simulink model "FullFMS_SIM_V0_1_8_R2025b"  (R2025b)
settings: Solver=FixedStepAuto  StopTime=inf  FixedStep=0.01  MaxStep=0.01  RelTol=1e-2
PreLoadFcn:
  | load("BUS_CONFIG_SIM.mat"); run("Param_SIM_V0_1_8.m")
libraries: opcualib x8
(part 2 of 2)

== stateflow chart FullFMS_SIM_V0_1_8_R2025b/Chart_SIM ==
  settings: updateMethod=DISCRETE  sampleTime=Ts_SIM
  state HD1_Ctrl [parallel]
    settings: executionOrder=2
    state Init
      entry: SimControl_50.SC_52_Profibus=true; SimControl_50.SC_55_PD_Sort=false; SimASi_50.SR_54_CRoute_Out=false;
      SimActuators_50.SA_50_Claw_Down=false; SimActuators_50.SA_50_Close_Claw=false; SimActuators_50.SA_50_Claw_2_Del=false; SimActuators_50.SA_50_Claw_2_Cart=false;
    state Ready
      entry: SimControl_50.SC_55_Initialization=true;
    state N1_StartMove
      entry: SimControl_50.SC_55_PD_Sort=false;
    state N2_LowerClaw
      entry: SimActuators_50.SA_50_Claw_Down=true;
    state N3_CloseClaw
      entry: SimActuators_50.SA_50_Close_Claw=true;
    state N3_Raise
      entry: SimActuators_50.SA_50_Claw_Down=false;
    state N4_Claw2Del
      entry: SimActuators_50.SA_50_Claw_2_Cart=false; SimActuators_50.SA_50_Claw_2_Del=true;
    state N5_LowerClaw2
      entry: SimActuators_50.SA_50_Claw_Down=true;
    state N6_Release
      entry: SimActuators_50.SA_50_Close_Claw=false;
    state N6_Raise
      entry: SimActuators_50.SA_50_Claw_Down=false;
    state N7_PDSort
      entry: SimControl_50.SC_55_PD_Sort=true;
    state N8_Claw2Cart
      entry: SimActuators_50.SA_50_Claw_2_Del=false; SimActuators_50.SA_50_Claw_2_Cart=true; Claw2CartCmd=true;
    state N9_CRouteOut
      entry: SimActuators_50.SA_50_Claw_2_Cart=false; Claw2CartCmd=false; RouteOut54=true; SimASi_50.SR_54_CRoute_Out=true;
      exit: RouteOut54=false; SimASi_50.SR_54_CRoute_Out=false; nCart = nCart + 1;
    (default) -> Init
    Init -> Ready : [SimSensors_50.SS_50_Claw_Cart && SimSensors_50.SS_50_Claw_High && ~SimSensors_50.SS_50_Part_in_Claw]
    N9_CRouteOut -> Ready : after(T_HD1_T1,sec)
    Ready -> N1_StartMove : [CRouteIn54 && CartAt29 && SimSensors_20.SS_29_Optic && ~SimSensors_60.SS_60_SPart]
    N1_StartMove -> N2_LowerClaw : [~SimControl_50.SC_55_PD_Sort && SimSensors_50.SS_50_Claw_Cart && SimSensors_50.SS_50_Claw_High && ~SimSensors_50.SS_50_Part_in_Claw]
    N2_LowerClaw -> N3_CloseClaw : [SimSensors_50.SS_50_Claw_Cart && SimSensors_50.SS_50_Claw_Low]
    N3_CloseClaw -> N3_Raise : [SimSensors_50.SS_50_Part_in_Claw]
    N3_Raise -> N4_Claw2Del : [SimSensors_50.SS_50_Claw_High && SimSensors_50.SS_50_Part_in_Claw && ~SimSensors_50.SS_50_Claw_Del]
    N4_Claw2Del -> N5_LowerClaw2 : [SimSensors_50.SS_50_Claw_Del && SimSensors_50.SS_50_Claw_High && SimSensors_50.SS_50_Part_in_Claw]
    N5_LowerClaw2 -> N6_Release : [SimSensors_50.SS_50_Claw_Del && SimSensors_50.SS_50_Claw_Low]
    N6_Release -> N6_Raise : [~SimSensors_50.SS_50_Part_in_Claw]
    N6_Raise -> N7_PDSort : [SimSensors_50.SS_50_Claw_Del && SimSensors_50.SS_50_Claw_High && ~SimSensors_50.SS_50_Part_in_Claw]
    N7_PDSort -> N8_Claw2Cart
    N8_Claw2Cart -> N9_CRouteOut : [SimSensors_50.SS_50_Claw_Cart]
  state HD1_Plant [parallel]
    settings: executionOrder=3
    state Vertical [parallel]
      settings: executionOrder=1
      state High
        entry: SimSensors_50.SS_50_Claw_High=true; SimSensors_50.SS_50_Claw_Low=false;
      state GoingDown
        entry: SimSensors_50.SS_50_Claw_High=false;
      state Low
        entry: SimSensors_50.SS_50_Claw_Low=true;
      state GoingUp
        entry: SimSensors_50.SS_50_Claw_Low=false;
      (default) -> High
      GoingUp -> High [order 1] : after(t_v_up,sec)
      High -> GoingDown : [SimActuators_50.SA_50_Claw_Down]
      GoingUp -> GoingDown [order 2] : [SimActuators_50.SA_50_Claw_Down]
      GoingDown -> Low [order 1] : after(t_v_down,sec)
      GoingDown -> GoingUp [order 2] : [~SimActuators_50.SA_50_Claw_Down]
      Low -> GoingUp : [~SimActuators_50.SA_50_Claw_Down]
    state Horizontal [parallel]
      settings: executionOrder=2
      state AtCart
        entry: SimSensors_50.SS_50_Claw_Cart=true; SimSensors_50.SS_50_Claw_Del=false;
      state ToDel
        entry: SimSensors_50.SS_50_Claw_Cart=false;
      state AtDel
        entry: SimSensors_50.SS_50_Claw_Del=true;
      state ToCart
        entry: SimSensors_50.SS_50_Claw_Del=false;
      (default) -> AtCart
      ToCart -> AtCart : after(t_h_cart,sec)
      AtCart -> ToDel : [SimActuators_50.SA_50_Claw_2_Del]
      ToDel -> AtDel : after(t_h_del,sec)
      AtDel -> ToCart : [SimActuators_50.SA_50_Claw_2_Cart]
    state Gripper [parallel]
      settings: executionOrder=3
      state Empty
        entry: SimSensors_50.SS_50_Part_in_Claw=false;
      state Gripping
      state Holding
        entry: SimSensors_50.SS_50_Part_in_Claw=true; cartPart=false;
      state Releasing
      (default) -> HD1_Plant.Gripper.Empty
      Releasing -> HD1_Plant.Gripper.Empty : after(t_grip,sec){SimSensors_60.SS_60_SPart = SimSensors_60.SS_60_SPart || SimSensors_50.SS_50_Claw_Del;}
      HD1_Plant.Gripper.Empty -> Gripping : [SimActuators_50.SA_50_Close_Claw && SimSensors_50.SS_50_Claw_Low && SimSensors_50.SS_50_Claw_Cart && PartOnCart]
      Gripping -> Holding : after(t_grip,sec)
      Holding -> Releasing : [~SimActuators_50.SA_50_Close_Claw && SimSensors_50.SS_50_Claw_Low]
  state SORT_Ctrl [parallel]
    entry: SimControl_60.SC_62_Profibus=false; SimControl_60.SC_65_Initialization=false; SimControl_60.SC_65_ID_1=false; SimControl_60.SC_65_ID_2=false; SimControl_60.SC_65_Part_Sorted=false;
    SimControl_60.SC_65_RBS_Output = (SORT_MODE == 1); SimControl_60.SC_65_RSB_Output = (SORT_MODE == 2); SimControl_60.SC_65_BRS_Output = (SORT_MODE == 3); SimControl_60.SC_65_BSR_Output = (SORT_MODE == 4); SimControl_60.SC_65_SRB_Output = (SORT_MODE == 5); SimControl_60.SC_65_SBR_Output = (SORT_MODE == 6);
    SimActuators_60.SA_60_Conveyor=false; SimActuators_60.SA_60_P1=false; SimActuators_60.SA_60_P2=false; SimActuators_60.SA_60_Identify=false; SimActuators_60.SA_61_Led_Start=false; SimActuators_60.SA_61_Led_Reset=false; SimActuators_60.SA_61_Led_Extra1=false; SimActuators_60.SA_61_Led_Extra2=false; SimActuators_60.SA_61_Panel_O4=false; SimActuators_60.SA_61_Panel_O5=false; SimActuators_60.SA_61_Panel_O6=false; SimActuators_60.SA_61_Panel_O7=false;
    FBSel = (SORT_MODE == 1 && SimControl_60.SC_65_RBS_Output) || (SORT_MODE == 2 && SimControl_60.SC_65_RSB_Output) || (SORT_MODE == 3 && SimControl_60.SC_65_BRS_Output) || (SORT_MODE == 4 && SimControl_60.SC_65_BSR_Output) || (SORT_MODE == 5 && SimControl_60.SC_65_SRB_Output) || (SORT_MODE == 6 && SimControl_60.SC_65_SBR_Output);
    settings: executionOrder=5
    state FB1_Init [parallel]
      settings: executionOrder=1
      state FB1_N2_Check
        entry: SimControl_60.SC_62_Profibus=true; FB1Init=false; SimControl_60.SC_65_Initialization=false;
      state FB1_N3_ClearPart
        entry: FB1Conv=true; FB1IDPin=true;
      state FB1_N1_InitOk
        entry: FB1Init=true; SimControl_60.SC_65_Initialization=true;
      (default) -> SORT_Ctrl.FB1_Init.FB1_N2_Check
      FB1_N3_ClearPart -> SORT_Ctrl.FB1_Init.FB1_N2_Check : [FB1Conv && SimSensors_60.SS_60_Part_Pass]{FB1Conv=false; FB1IDPin=false;}
      SORT_Ctrl.FB1_Init.FB1_N1_InitOk -> SORT_Ctrl.FB1_Init.FB1_N2_Check : [SimSensors_60.SS_61_Reset]{FB1Conv=false; FB1IDPin=false; TrigConv=false; Lever1=false; Lever2=false; PinSort=false; PartDel=false;}
      SORT_Ctrl.FB1_Init.FB1_N2_Check -> SORT_Ctrl.FB1_Init.FB1_N1_InitOk [order 1] : [SimControl_60.SC_62_Profibus && ~FB1Conv && ~SimSensors_60.SS_60_SPart && ~SimSensors_60.SS_60_SInd && ~SimSensors_60.SS_60_SPhoto && ~SimSensors_60.SS_60_Part_Pass]
      SORT_Ctrl.FB1_Init.FB1_N2_Check -> FB1_N3_ClearPart [order 2] : [SimSensors_60.SS_60_SPart || SimSensors_60.SS_60_SInd || SimSensors_60.SS_60_SPhoto]
    state FB4_9_Sort [parallel]
      settings: executionOrder=2
      state OB1_N4_9_Select
      state N1_StartConv
        entry: TrigConv=true; SimControl_60.SC_65_ID_1=false; SimControl_60.SC_65_ID_2=false;
      state N2_Identify
        en, du: if SimSensors_60.SS_60_SInd, SimControl_60.SC_65_ID_1=false; SimControl_60.SC_65_ID_2=true;
        elseif SimSensors_60.SS_60_SPhoto, SimControl_60.SC_65_ID_1=true; SimControl_60.SC_65_ID_2=true;
        else, SimControl_60.SC_65_ID_1=true; SimControl_60.SC_65_ID_2=false; end
      state N3_SelectLever
        entry: cID = 0;
        if SimControl_60.SC_65_ID_1 && SimControl_60.SC_65_ID_2, cID = 1; elseif SimControl_60.SC_65_ID_1, cID = 2; elseif SimControl_60.SC_65_ID_2, cID = 3; end
        Lever1 = (cID == SORT_MAP(SORT_MODE,1)); Lever2 = (cID == SORT_MAP(SORT_MODE,2)); PassStr = (cID == SORT_MAP(SORT_MODE,3));
        during: if (Lever1 && SimSensors_60.SS_60_SL1_Fwd) || (Lever2 && SimSensors_60.SS_60_SL2_Fwd) || (PassStr && SimSensors_60.SS_60_SL1_Bck && SimSensors_60.SS_60_SL2_Bck), PinSort = true; end
      state N4_PartDel
        entry: PartDel=true; Lever1=false;
        if SORT_MODE ~= 3, Lever2=false; end
      state N5_ResetNext
        entry: TrigConv=false; PinSort=false; PartDel=false; Lever1=false; Lever2=false; PassStr=false;
      (default) -> OB1_N4_9_Select
      N5_ResetNext -> OB1_N4_9_Select
      OB1_N4_9_Select -> N1_StartConv : [FB1Init && FBSel && SimControl_50.SC_55_PD_Sort && SimSensors_50.SS_50_Claw_Del]
      N1_StartConv -> N2_Identify
      N2_Identify -> N3_SelectLever : after(T_SORT_ID - Ts_SIM,sec)
      N3_SelectLever -> N4_PartDel : [SimSensors_60.SS_60_Part_Pass]
      N4_PartDel -> N5_ResetNext
    state OB1_N10_11 [parallel]
      settings: executionOrder=3
      state N10_Wait
        entry: SimControl_60.SC_65_Part_Sorted=false;
      state N10_PartPass
      state N11_PartSorted
        entry: SimControl_60.SC_65_Part_Sorted=true;
      (default) -> N10_Wait
      N11_PartSorted -> N10_Wait : after(T_SORT_T7,sec)
      N10_Wait -> N10_PartPass : [SimSensors_60.SS_60_Part_Pass]
      N10_PartPass -> N11_PartSorted : [~SimSensors_60.SS_60_Part_Pass]
    state FB3_Actuators [parallel]
      settings: executionOrder=4
      state FB3_Map
        during: ConvOn60 = SimSensors_60.SS_61_Key_Pos && (TrigConv || FB1Conv); SimActuators_60.SA_60_Conveyor = ConvOn60;
        SimActuators_60.SA_60_P1 = SimSensors_60.SS_61_Key_Pos && Lever1; SimActuators_60.SA_60_P2 = SimSensors_60.SS_61_Key_Pos && Lever2;
        SimActuators_60.SA_60_Identify = SimSensors_60.SS_61_Key_Pos && (PinSort || FB1IDPin);
        SimActuators_60.SA_61_Led_Start = SimSensors_60.SS_61_Key_Pos && FB1Init; SimActuators_60.SA_61_Led_Reset = SimSensors_60.SS_61_Key_Pos && SimSensors_60.SS_61_Reset;
        SimActuators_60.SA_61_Led_Extra1 = SimControl_60.SC_65_Part_Sorted; SimActuators_60.SA_61_Led_Extra2 = false;
        SimActuators_60.SA_61_Panel_O4 = false; SimActuators_60.SA_61_Panel_O5 = false; SimActuators_60.SA_61_Panel_O6 = false; SimActuators_60.SA_61_Panel_O7 = false;
      (default) -> SORT_Ctrl.FB3_Actuators.FB3_Map
  state SORT_Plant [parallel]
    entry: SimSensors_60.SS_60_SPart=false; SimSensors_60.SS_60_SInd=false; SimSensors_60.SS_60_SPhoto=false; SimSensors_60.SS_60_Part_Pass=false;
    SimSensors_60.SS_60_SL1_Bck=true; SimSensors_60.SS_60_SL1_Fwd=false; SimSensors_60.SS_60_SL2_Bck=true; SimSensors_60.SS_60_SL2_Fwd=false;
    SimSensors_60.SS_61_Key_Pos=true; SimSensors_60.SS_61_Start=false; SimSensors_60.SS_61_Stop=false; SimSensors_60.SS_61_Reset=false;
    SimSensors_60.SS_61_Panel_I4=false; SimSensors_60.SS_61_Panel_I5=false; SimSensors_60.SS_61_Panel_I6=false; SimSensors_60.SS_61_Panel_I7=false;
    settings: executionOrder=4
    state Part [parallel]
      settings: executionOrder=1
      state Empty
        entry: SimSensors_60.SS_60_Part_Pass=false;
      state AtEntry
        entry: sortColor = PART_COLORS(min(nSortIn+1, numel(PART_COLORS))); nSortIn = nSortIn + 1;
      state ToStopper
        entry: xSort = 0;
        during: if ConvOn60, xSort = xSort + Ts_SIM; end
        SimSensors_60.SS_60_SPart = xSort < t_s_spart_off;
        if xSort >= t_s_photo, SimSensors_60.SS_60_SPhoto = (sortColor ~= 2); end
        if xSort >= t_s_ind, SimSensors_60.SS_60_SInd = (sortColor == 3); end
      state AtStopper
      state Released
        entry: xSort = 0;
        if SimSensors_60.SS_60_SL1_Fwd, sortExit = 1; elseif SimSensors_60.SS_60_SL2_Fwd, sortExit = 2; else, sortExit = 3; end
        during: if ConvOn60, xSort = xSort + Ts_SIM; end
        if xSort >= t_s_ind_off, SimSensors_60.SS_60_SInd = false; end
        if xSort >= t_s_photo_off, SimSensors_60.SS_60_SPhoto = false; end
      state PartPass
        entry: SimSensors_60.SS_60_Part_Pass = true; SimSensors_60.SS_60_SInd = false; SimSensors_60.SS_60_SPhoto = false; nDone = nDone + 1;
      (default) -> SORT_Plant.Part.Empty
      PartPass -> SORT_Plant.Part.Empty : after(t_s_pp,sec)
      SORT_Plant.Part.Empty -> AtEntry : [SimSensors_60.SS_60_SPart]
      AtEntry -> ToStopper : [SimActuators_60.SA_60_Conveyor]
      ToStopper -> AtStopper : [xSort >= t_s_ind]
      AtStopper -> Released : [SimActuators_60.SA_60_Identify && SimActuators_60.SA_60_Conveyor]
      Released -> PartPass : [(sortExit == 1 && xSort >= t_s_pass1) || (sortExit == 2 && xSort >= t_s_pass2) || (sortExit == 3 && xSort >= t_s_pass3)]
    state Lever1 [parallel]
      settings: executionOrder=2
      state SL1_Bck
        entry: SimSensors_60.SS_60_SL1_Bck=true; SimSensors_60.SS_60_SL1_Fwd=false;
      state SL1_ToFwd
        entry: SimSensors_60.SS_60_SL1_Bck=false;
      state SL1_Fwd
        entry: SimSensors_60.SS_60_SL1_Fwd=true;
      state SL1_ToBck
        entry: SimSensors_60.SS_60_SL1_Fwd=false;
      (default) -> SL1_Bck
      SL1_ToBck -> SL1_Bck [order 1] : after(t_sl1_bck,sec)
      SL1_Bck -> SL1_ToFwd : [SimActuators_60.SA_60_P1]
      SL1_ToBck -> SL1_ToFwd [order 2] : [SimActuators_60.SA_60_P1]
      SL1_ToFwd -> SL1_Fwd [order 1] : after(t_sl1_fwd,sec)
      SL1_ToFwd -> SL1_ToBck [order 2] : [~SimActuators_60.SA_60_P1]
      SL1_Fwd -> SL1_ToBck : [~SimActuators_60.SA_60_P1]
    state Lever2 [parallel]
      settings: executionOrder=3
      state SL2_Bck
        entry: SimSensors_60.SS_60_SL2_Bck=true; SimSensors_60.SS_60_SL2_Fwd=false;
      state SL2_ToFwd
        entry: SimSensors_60.SS_60_SL2_Bck=false;
      state SL2_Fwd
        entry: SimSensors_60.SS_60_SL2_Fwd=true;
      state SL2_ToBck
        entry: SimSensors_60.SS_60_SL2_Fwd=false;
      (default) -> SL2_Bck
      SL2_ToBck -> SL2_Bck [order 1] : after(t_sl2_bck,sec)
      SL2_Bck -> SL2_ToFwd : [SimActuators_60.SA_60_P2]
      SL2_ToBck -> SL2_ToFwd [order 2] : [SimActuators_60.SA_60_P2]
      SL2_ToFwd -> SL2_Fwd [order 1] : after(t_sl2_fwd,sec)
      SL2_ToFwd -> SL2_ToBck [order 2] : [~SimActuators_60.SA_60_P2]
      SL2_Fwd -> SL2_ToBck : [~SimActuators_60.SA_60_P2]
  state TEST_Ctrl [parallel]
    entry: SimControl_70.SC_72_Profibus=false; SimControl_70.SC_75_Initialization=false; SimControl_70.SC_75_RQ_Delivery1=false; SimControl_70.SC_75_ID_Delivery1=false; SimControl_70.SC_75_RQ_Delivery2=false; SimControl_70.SC_75_ID_Delivery2=false; SimControl_70.SC_75_Part_Del=false; SimControl_70.SC_75_RQ_Part_Del=false; SimControl_70.SC_75_RQ_Wrong=false;
    SimControl_70.SC_75_Identified = (TEST_MODE == 1); SimControl_70.SC_75_Requested = (TEST_MODE == 2); SimControl_70.SC_75_Identified80 = (TEST_MODE == 1); SimControl_70.SC_75_Requested80 = (TEST_MODE == 2);
    SimActuators_70.SA_70_Elev_Down=false; SimActuators_70.SA_70_Elev_Up=false; SimActuators_70.SA_70_Eject_Part=false; SimActuators_70.SA_70_Air_On=false; SimActuators_70.SA_71_Led_Start=false; SimActuators_70.SA_71_Led_Reset=false; SimActuators_70.SA_71_Led_Extra1=false; SimActuators_70.SA_71_Led_Extra2=false; SimActuators_70.SA_71_Panel_O4=false; SimActuators_70.SA_71_Panel_O5=false; SimActuators_70.SA_71_Panel_O6=false; SimActuators_70.SA_71_Panel_O7=false;
    SimASi_70.SR_73_TestCartID=0; SimASi_70.SR_74_Request=false; SimASi_70.SR_74_No_Cart=true; SimASi_70.SR_74_Cart_Full=false; SimASi_70.SR_74_CRoute_Out=false; SimASi_70.SR_74_CRoute_In=false;
    settings: executionOrder=6
    state FB1_Init70 [parallel]
      settings: executionOrder=1
      state FB1_N2_N3_Check
        entry: SimControl_70.SC_72_Profibus=true; FB1Init70=false; SimControl_70.SC_75_Initialization=false;
        during: FB1ElevDown70 = ~ElevLow70;
      state FB1_N3_PistonPulse
        entry: FB1PistAdv70=true;
      state FB1_N1_N4_InitOk
        entry: FB1Init70=true; SimControl_70.SC_75_Initialization=true; FB1ElevDown70=false; FB1PistAdv70=false;
      (default) -> TEST_Ctrl.FB1_Init70.FB1_N2_N3_Check
      FB1_N3_PistonPulse -> TEST_Ctrl.FB1_Init70.FB1_N2_N3_Check : after(T_TEST_T1,sec){FB1PistAdv70=false;}
      FB1_N1_N4_InitOk -> TEST_Ctrl.FB1_Init70.FB1_N2_N3_Check : [SimSensors_70.SS_71_Reset]{IdenDel=false; IdenProc=false; EjectProc=false; ReturnElev=false; ReqDel=false; IdenColor=false; PartOk=false; EjectOk=false; PartDiff=false; EjectBad=false;}
      TEST_Ctrl.FB1_Init70.FB1_N2_N3_Check -> FB1_N1_N4_InitOk [order 1] : [~PartIn70 && ElevLow70 && PistBck70 && DistInit85]
      TEST_Ctrl.FB1_Init70.FB1_N2_N3_Check -> FB1_N3_PistonPulse [order 2] : [ElevLow70 && PartIn70]
    state FB4_Identified [parallel]
      settings: executionOrder=2
      state OB1_N4_Off
      state FB4_Wait
      state N1_StartID
        entry: IdenDel=true; idA70=false; idB70=false; PartDel70=false; RQPartDel70=false;
      state N2_N3_Raise
        en, du: if PartIn70 && ElevLow70 && SInd70, idB70 = true; end
        FB4ElevUp = PartIn70 && PistBck70 && ArmMag80;
      state N4_Identify
        entry: IdenProc=true; FB4ElevUp=true;
        en, du: if ~idB70, idA70 = true; if Height70, idB70 = true; end; end
      state N5_EjectWaitCart
        entry: IdenProc=false; EjectProc=true; FB4ElevUp=true;
      state N5_EjectPush
        entry: FB4PistFwd=true; FB4Air=true;
      state N5_EjectEnd
        entry: FB4PistFwd=false; FB4Air=false;
        en, du: FB4CartFull = CartStat24 && Optic24 && ~PistBck24;
      state N6_ReturnElev
        entry: EjectProc=false; ReturnElev=true; FB4ElevUp=false; FB4CartFull=false; FB4ElevDown=ArmMag80;
      state N6_PartDel
        entry: FB4ElevDown=false; PartDel70=true; ReturnElev=false;
      (default) -> OB1_N4_Off
      OB1_N4_Off -> TEST_Ctrl.FB4_Identified.FB4_Wait : [FB1Init70 && SimControl_70.SC_75_Identified]
      N6_PartDel -> TEST_Ctrl.FB4_Identified.FB4_Wait
      TEST_Ctrl.FB4_Identified.FB4_Wait -> N1_StartID : [PartIn70]
      N1_StartID -> TEST_Ctrl.FB4_Identified.N2_N3_Raise
      TEST_Ctrl.FB4_Identified.N2_N3_Raise -> N4_Identify : [ElevHigh70 && FB4ElevUp]
      N4_Identify -> N5_EjectWaitCart : after(T_TEST_T2,sec)
      N5_EjectWaitCart -> N5_EjectPush : [~PistBck24 && CartStat24 && ~Optic24]
      N5_EjectPush -> N5_EjectEnd [order 1] : [Optic24]
      N5_EjectPush -> N5_EjectEnd [order 2] : after(T_TEST_T3,sec)
      N5_EjectEnd -> N6_ReturnElev : [PistBck70 && ~PartIn70 && Optic24]
      N6_ReturnElev -> N6_PartDel : [ElevLow70]
    state FB5_Requested [parallel]
      settings: executionOrder=3
      state OB1_N5_Off
      state FB5_Wait
      state N1_StartReq
        entry: ReqDel=true; PartDiff=false; idA70=false; idB70=false; PartDel70=false; RQPartDel70=false; RQWrong70=false;
      state N2_N3_Raise
        en, du: if PartIn70 && ElevLow70 && SInd70, idB70 = true; end
        FB5ElevUp = PartIn70 && PistBck70 && ArmMag80 && ~PartDiff;
      state N4_ColorWindow
        entry: IdenColor=true; FB5ElevUp=true;
        en, du: if ~idB70, idA70 = true; if Height70, idB70 = true; end; end
      state N4_ColorHold
      state N5_Compare
        entry: IdenColor=false; FB5ElevUp=false;
        if (idA70 == RQ1_70) && (idB70 == RQ2_70), PartOk=true; EjectOk=true;
        else, PartDiff=true; EjectBad=true; end
      state N6_EjectWaitCart
      state N6_EjectPush
        entry: FB5PistFwd1=true; FB5Air=true;
      state N6_EjectEnd
        entry: FB5PistFwd1=false; FB5Air=false;
        en, du: FB5CartFull = CartStat24 && Optic24 && ~PistBck24;
      state N7_ReturnElev
        entry: EjectOk=false; ReturnElev=true; FB5CartFull=false; FB5ElevDown1=ArmMag80;
      state N7_RQPartDel
        entry: FB5ElevDown1=false; RQPartDel70=true; ReturnElev=false; PartOk=false;
      state N10_ResetReq
        entry: ReqDel=false;
      state N8_DownBad
        entry: FB5ElevDown2=ArmMag80;
      state N8_EjectBad
        entry: FB5ElevDown2=false; FB5PistFwd2=true;
      state N8_WaitBack
        entry: FB5PistFwd2=false;
      state N9_RQWrong
        entry: EjectBad=false; RQWrong70=true;
      (default) -> TEST_Ctrl.FB5_Requested.OB1_N5_Off
      TEST_Ctrl.FB5_Requested.OB1_N5_Off -> TEST_Ctrl.FB5_Requested.FB5_Wait : [FB1Init70 && SimControl_70.SC_75_Requested]
      N10_ResetReq -> TEST_Ctrl.FB5_Requested.FB5_Wait
      N9_RQWrong -> TEST_Ctrl.FB5_Requested.FB5_Wait
      TEST_Ctrl.FB5_Requested.FB5_Wait -> N1_StartReq : [PartIn70]
      N1_StartReq -> TEST_Ctrl.FB5_Requested.N2_N3_Raise
      TEST_Ctrl.FB5_Requested.N2_N3_Raise -> N4_ColorWindow : [ElevHigh70 && FB5ElevUp]
      N4_ColorWindow -> N4_ColorHold : after(T_TEST_T8,sec)
      N4_ColorHold -> N5_Compare : after(T_TEST_T2 - T_TEST_T8,sec)
      N5_Compare -> N6_EjectWaitCart [order 1] : [PartOk]
      N5_Compare -> N8_DownBad [order 2] : [PartDiff]
      N6_EjectWaitCart -> N6_EjectPush : [~PistBck24 && CartStat24 && ~Optic24]
      N6_EjectPush -> N6_EjectEnd [order 1] : [Optic24]
      N6_EjectPush -> N6_EjectEnd [order 2] : after(T_TEST_T5,sec)
      N6_EjectEnd -> N7_ReturnElev : [PistBck70 && ~PartIn70 && Optic24]
      N7_ReturnElev -> N7_RQPartDel : [ElevLow70]
      N7_RQPartDel -> N10_ResetReq
      N8_DownBad -> N8_EjectBad : [ElevLow70]
      N8_EjectBad -> N8_WaitBack : after(T_TEST_T6,sec)
      N8_WaitBack -> N9_RQWrong : [PistBck70 && ~PartIn70]
    state OB1_N6_Routing [parallel]
      settings: executionOrder=4
      state OB1_N6_Wait
      state OB1_N6_T7_CRouteOut
        entry: SimASi_70.SR_74_CRoute_Out=true; RouteOut74=true;
      state OB1_N6_Hold
        entry: SimASi_70.SR_74_CRoute_Out=false; RouteOut74=false;
      (default) -> OB1_N6_Wait
      OB1_N6_Hold -> OB1_N6_Wait : [~PartDel70 && ~RQPartDel70]
      OB1_N6_Wait -> OB1_N6_T7_CRouteOut : [PartDel70 || RQPartDel70]
      OB1_N6_T7_CRouteOut -> OB1_N6_Hold : after(T_TEST_T7,sec)
    state FB3_OB1_Map [parallel]
      settings: executionOrder=5
      state FB3_Map
        during: ElevUp70 = KeyPos71 && (FB4ElevUp || FB5ElevUp);
        ElevDown70 = KeyPos71 && (FB1ElevDown70 || FB4ElevDown || FB5ElevDown1 || FB5ElevDown2);
        Eject70 = KeyPos71 && (FB1PistAdv70 || FB4PistFwd || FB5PistFwd1 || FB5PistFwd2);
        Air70 = KeyPos71 && (FB4Air || FB5Air);
        SimActuators_70.SA_70_Elev_Up = ElevUp70; SimActuators_70.SA_70_Elev_Down = ElevDown70; SimActuators_70.SA_70_Eject_Part = Eject70; SimActuators_70.SA_70_Air_On = Air70;
        NoCart74 = ~CartStat24; CartFull74 = (FB4CartFull && TEST_MODE == 1) || (FB5CartFull && TEST_MODE == 2) || (CartStat24 && Optic24);
        SimASi_70.SR_74_No_Cart = NoCart74; SimASi_70.SR_74_Cart_Full = CartFull74; CRouteIn80 = CRouteIn74;
        SimActuators_70.SA_71_Led_Start = KeyPos71 && FB1Init70; SimActuators_70.SA_71_Led_Extra1 = NoCart74; SimActuators_70.SA_71_Led_Extra2 = CartFull74;
        SimControl_70.SC_75_ID_Delivery1 = idA70; SimControl_70.SC_75_ID_Delivery2 = idB70; SimControl_70.SC_75_Part_Del = PartDel70;
        SimControl_70.SC_75_RQ_Part_Del = RQPartDel70; SimControl_70.SC_75_RQ_Wrong = RQWrong70;
      (default) -> TEST_Ctrl.FB3_OB1_Map.FB3_Map
  state TEST_Plant [parallel]
    entry: KeyPos71=true; ElevLow70=true; PistBck70=true;
    SimSensors_70.SS_71_Key_Pos=true; SimSensors_70.SS_71_Start=false; SimSensors_70.SS_71_Stop=false; SimSensors_70.SS_71_Reset=false;
    SimSensors_70.SS_71_Panel_I4=false; SimSensors_70.SS_71_Panel_I5=false; SimSensors_70.SS_71_Panel_I6=false; SimSensors_70.SS_71_Panel_I7=false;
    settings: executionOrder=7
    state Elevator [parallel]
      settings: executionOrder=1
      state Elev_Low
        entry: ElevLow70=true; ElevHigh70=false; SInd70 = PartIn70 && testColor == 3; SStation70=false;
      state Elev_GoingUp
        entry: tElev = 0;
        during: tElev = tElev + Ts_SIM; ElevLow70 = tElev < t_t_up_lowoff;
        SInd70 = (PartIn70 && testColor == 3 && tElev < t_t_metal_off) || (tElev >= t_t_up_ind && tElev < t_t_up_ind + 0.15);
        SStation70 = tElev >= t_t_up_sst && tElev < t_t_up_sst + 0.22;
        Height70 = PartIn70 && testColor ~= 2 && tElev >= t_t_up - t_t_height_pre;
      state Elev_High
        entry: ElevHigh70=true; ElevLow70=false; SInd70=false; SStation70=false; Height70 = PartIn70 && testColor ~= 2;
      state Elev_GoingDown
        entry: tElev = 0; Height70=false;
        during: tElev = tElev + Ts_SIM; ElevHigh70 = tElev < t_t_down_highoff;
        SStation70 = tElev >= t_t_down_sst && tElev < t_t_down_sst + 0.27;
        SInd70 = (tElev >= t_t_down_ind && tElev < t_t_down_ind + 0.18) || (PartIn70 && testColor == 3 && tElev >= t_t_down - 0.3);
      (default) -> Elev_Low
      Elev_GoingDown -> Elev_Low [order 1] : [tElev >= t_t_down]
      Elev_Low -> Elev_GoingUp : [ElevUp70 && ~ElevDown70]
      Elev_GoingDown -> Elev_GoingUp [order 2] : [ElevUp70 && ~ElevDown70]
      Elev_GoingUp -> Elev_High [order 1] : [tElev >= t_t_up]
      Elev_GoingUp -> Elev_GoingDown [order 2] : [ElevDown70]
      Elev_High -> Elev_GoingDown : [ElevDown70]
    state SlideToCart [parallel]
      settings: executionOrder=3
      state Slide_Empty
      state Slide_Moving
        entry: PartToCart=false;
      state Slide_OnCart
        entry: if CartStat24, cartPart=true; end
      (default) -> Slide_Empty
      Slide_OnCart -> Slide_Empty
      Slide_Empty -> Slide_Moving : [PartToCart]
      Slide_Moving -> Slide_OnCart : after(t_t_ej_cart - t_t_ej_spart,sec)
    state Sensors_Out [parallel]
      settings: executionOrder=4
      state S70_Map
        en, du: SimSensors_70.SS_70_SPart = PartIn70; SimSensors_70.SS_70_Elev_Low = ElevLow70; SimSensors_70.SS_70_Elev_High = ElevHigh70;
        SimSensors_70.SS_70_SInductive = SInd70; SimSensors_70.SS_70_SPart_Height = Height70; SimSensors_70.SS_70_Pist_Bck = PistBck70;
        SimSensors_70.SS_70_SStation = SStation70;
      (default) -> S70_Map
    state Piston [parallel]
      settings: executionOrder=2
      state Pist_Back
        entry: PistBck70=true;
      state Pist_Fwd
        entry: tPist = 0;
        during: tPist = tPist + Ts_SIM; PistBck70 = tPist < t_t_pist_fwd;
        if PartIn70 && tPist >= t_t_ej_spart
        PartIn70 = false; Height70 = false; SInd70 = false;
        if ElevHigh70, PartToCart = true; else, nReject = nReject + 1; end
        end
      state Pist_Return
        entry: PistBck70=false;
      (default) -> Pist_Back
      Pist_Return -> Pist_Back : after(t_t_pist_back,sec)
      Pist_Back -> Pist_Fwd : [Eject70]
      Pist_Fwd -> Pist_Return : [~Eject70]
  state DIST_Ctrl [parallel]
    entry: SimControl_80.SC_82_Profibus=false; SimControl_80.SC_85_Initialization=false; SimControl_80.SC_85_Start=false; SimControl_80.SC_85_Part_Del=false;
    SimControl_80.SC_85_Single = (DIST_MODE == 1); SimControl_80.SC_85_Continuous = (DIST_MODE == 2); SimControl_80.SC_85_Counted = (DIST_MODE == 3);
    SimControl_80.SC_85_Part_Mag=false; SimControl_80.SC_83_RQ_Parts = RQ_PARTS; SimControl_80.SC_86_Mag_Parts = 0; SimControl_80.SC_87_RQ_MParts = 0;
    SimActuators_80.SA_80_Pist_Adv=false; SimActuators_80.SA_80_Suction_On=false; SimActuators_80.SA_80_Suction_Off=false; SimActuators_80.SA_80_Arm_2_Del=false; SimActuators_80.SA_80_Arm_2_Mag=false; SimActuators_80.SA_81_Led_Start=false; SimActuators_80.SA_81_Led_Reset=false; SimActuators_80.SA_81_Led_Extra1=false; SimActuators_80.SA_81_Led_Extra2=false; SimActuators_80.SA_81_Panel_O4=false; SimActuators_80.SA_81_Panel_O5=false; SimActuators_80.SA_81_Panel_O6=false; SimActuators_80.SA_81_Panel_O7=false;
    settings: executionOrder=9
    state FB1_Init80 [parallel]
      settings: executionOrder=1
      state FB1_N2_Check
        entry: SimControl_80.SC_82_Profibus=true; DistInit85=false; SimControl_80.SC_85_Initialization=false;
      state FB1_N3_N4_EmptyMag
        entry: DistInit85=false;
      state FB1_N5_ArmToMag
        en, du: FB1A2M2_80 = ~ArmMag80;
      state FB1_N1_N5_InitOk
        entry: FB1A2M2_80=false; DistInit85=true; SimControl_80.SC_85_Initialization=true;
      (default) -> DIST_Ctrl.FB1_Init80.FB1_N2_Check
      FB1_N1_N5_InitOk -> DIST_Ctrl.FB1_Init80.FB1_N2_Check : [SimSensors_80.SS_81_Reset]
      DIST_Ctrl.FB1_Init80.FB1_N2_Check -> FB1_N5_ArmToMag [order 1] : [MagEmpty80 || MagFull80]{FB1MagEmpty80 = MagEmpty80; FB1MagFull80 = MagFull80;}
      DIST_Ctrl.FB1_Init80.FB1_N2_Check -> FB1_N3_N4_EmptyMag [order 2] : [~MagEmpty80 && ~MagFull80]
      FB1_N5_ArmToMag -> FB1_N1_N5_InitOk : [ArmMag80 && SimControl_80.SC_82_Profibus]
    state OB1_N4_N6_Counter [parallel]
      settings: executionOrder=2
      state OB1_N4_C1
        en, du: if MagFull80 && ~prevMagFull80, cnt80 = cnt80 + 1; end
        if PistFwd80 && ~prevPistFwd80, cnt80 = max(cnt80 - 1, 0); end
        if MagFull80, tMagFull = tMagFull + Ts_SIM; else, tMagFull = 0; end
        if tMagFull >= T_DIST_T1 && tMagFull < T_DIST_T1 + Ts_SIM, cnt80 = 9; end
        if PistBck80 && MagEmpty80, tMagEmpty = tMagEmpty + Ts_SIM; else, tMagEmpty = 0; end
        if tMagEmpty >= T_DIST_T2, cnt80 = 0; end
        prevMagFull80 = MagFull80; prevPistFwd80 = PistFwd80; PartinMag80 = cnt80 > 0;
        SimControl_80.SC_85_Part_Mag = PartinMag80; SimControl_80.SC_86_Mag_Parts = cnt80; SimControl_80.SC_87_RQ_MParts = cnt87;
      (default) -> OB1_N4_C1
    state FB4_Single [parallel]
      settings: executionOrder=4
      state OB1_N7_Off
      state FB4_Wait
      state FB4_N1_SingleOn
        entry: D4On=true;
      state D4_A2D_1
        en, du: D4A2D1 = ~ArmDel80 && ElevLow70 && ~PartIn70;
      state D4_PistFwd
        entry: D4A2D1=false; D4PistFwd=true;
      state D4_Transport
        entry: D4Transport=true; D4PistFwd=false;
      state D4_A2M_1
        en, du: D4A2M1 = ~ArmMag80;
      state D4_SuctOn
        entry: D4A2M1=false; D4SuctOn=true;
      state D4_PartStuck
        entry: D4PartStuckM=true;
      state D4_A2D_2
        en, du: D4A2D2 = ~ArmDel80 && ElevLow70 && ~PartIn70;
      state D4_SuctOff
        entry: D4A2D2=false; D4SuctOn=false;
        en, du: D4SuctOff = PartStuck80;
      state D4_PartDel
        entry: D4SuctOff=false; D4PartDel=true; D4Transport=false; D4PartStuckM=false;
      state D4_A2M_2
        en, du: D4A2M2 = ~ArmMag80;
      state D4_Reset
        entry: D4A2M2=false; D4On=false; D4PartDel=false;
      (default) -> DIST_Ctrl.FB4_Single.OB1_N7_Off
      DIST_Ctrl.FB4_Single.OB1_N7_Off -> DIST_Ctrl.FB4_Single.FB4_Wait : [DistInit85 && SimControl_80.SC_85_Single]
      D4_Reset -> DIST_Ctrl.FB4_Single.FB4_Wait
      DIST_Ctrl.FB4_Single.FB4_Wait -> FB4_N1_SingleOn : [(SimSensors_80.SS_81_Start || SimControl_80.SC_85_Start || RQWrong70 || (CRouteIn80 && KeyPos81)) && ElevLow70 && ~PartIn70 && PartinMag80]
      FB4_N1_SingleOn -> D4_A2D_1
      D4_A2D_1 -> D4_PistFwd : [ArmDel80 && PistBck80]
      D4_PistFwd -> D4_Transport : [PistFwd80]
      D4_Transport -> D4_A2M_1
      D4_A2M_1 -> D4_SuctOn : [ArmMag80]
      D4_SuctOn -> D4_PartStuck : [PartStuck80]
      D4_PartStuck -> D4_A2D_2
      D4_A2D_2 -> D4_SuctOff : [ArmDel80]
      D4_SuctOff -> D4_PartDel : [~PartStuck80]
      D4_PartDel -> D4_A2M_2
      D4_A2M_2 -> D4_Reset : [ArmMag80]
    state FB5_Continuous [parallel]
      settings: executionOrder=5
      state OB1_N8_Off
      state FB5_Wait
      state FB5_N1_AutoOn
        entry: D5On=true;
      state D5_A2D_1
        en, du: D5A2D1 = ~ArmDel80 && ElevLow70 && ~PartIn70;
      state D5_PistFwd
        entry: D5A2D1=false; D5PistFwd=true;
      state D5_Transport
        entry: D5Transport=true; D5PistFwd=false;
      state D5_A2M_1
        en, du: D5A2M1 = ~ArmMag80;
      state D5_SuctOn
        entry: D5A2M1=false; D5SuctOn=true;
      state D5_PartStuck
        entry: D5PartStuckM=true;
      state D5_A2D_2
        en, du: D5A2D2 = ~ArmDel80 && ElevLow70 && ~PartIn70;
      state D5_SuctOff
        entry: D5A2D2=false; D5SuctOn=false;
        en, du: D5SuctOff = PartStuck80;
      state D5_PartDel
        entry: D5SuctOff=false; D5Transport=false; D5PartStuckM=false; D5PartDelEdge=true;
      state D5_N3_T3
        entry: D5PartDelEdge=false;
      state D5_N3_A2M_2
        en, du: D5A2M2 = ~ArmMag80;
      state D5_N4_Reset
        entry: D5A2M2=false; D5On=false;
      (default) -> OB1_N8_Off
      OB1_N8_Off -> DIST_Ctrl.FB5_Continuous.FB5_Wait : [DistInit85 && SimControl_80.SC_85_Continuous]
      D5_N4_Reset -> DIST_Ctrl.FB5_Continuous.FB5_Wait
      DIST_Ctrl.FB5_Continuous.FB5_Wait -> FB5_N1_AutoOn : [(SimSensors_80.SS_81_Start || SimControl_80.SC_85_Start || (CRouteIn80 && KeyPos81)) && ElevLow70 && ~PartIn70 && PartinMag80]
      FB5_N1_AutoOn -> D5_A2D_1
      D5_A2D_1 -> D5_PistFwd : [ArmDel80 && PistBck80]
      D5_PartDel -> D5_PistFwd [order 1] : [~MagEmpty80 && PistBck80 && ArmDel80]{D5PartDelEdge=false; D5PistFwd=true;}
      D5_PistFwd -> D5_Transport : [PistFwd80]
      D5_Transport -> D5_A2M_1
      D5_A2M_1 -> D5_SuctOn : [ArmMag80]
      D5_SuctOn -> D5_PartStuck : [PartStuck80]
      D5_PartStuck -> D5_A2D_2
      D5_A2D_2 -> D5_SuctOff : [ArmDel80]
      D5_SuctOff -> D5_PartDel : [~PartStuck80]
      D5_PartDel -> D5_N3_T3 [order 2] : [MagEmpty80 && PistBck80 && ArmDel80]
      D5_N3_T3 -> D5_N3_A2M_2 : after(T_DIST_T3,sec)
      D5_N3_A2M_2 -> D5_N4_Reset : [ArmMag80]
    state FB6_Counted [parallel]
      settings: executionOrder=6
      state OB1_N9_Off
      state FB6_Wait
      state FB6_N1_N2_LoadC2
        entry: cnt87 = RQ_PARTS + 1; D6On = cnt87 > 0;
      state D6_A2D_1
        en, du: D6A2D1 = ~ArmDel80 && ElevLow70 && ~PartIn70;
      state D6_PistFwd
        entry: D6A2D1=false; D6PistFwd=true;
      state D6_Transport
        entry: D6Transport=true; D6PistFwd=false;
      state D6_A2M_1
        en, du: D6A2M1 = ~ArmMag80;
      state D6_SuctOn
        entry: D6A2M1=false; D6SuctOn=true;
      state D6_PartStuck
        entry: D6PartStuckM=true;
      state D6_A2D_2
        en, du: D6A2D2 = ~ArmDel80 && ElevLow70 && ~PartIn70;
      state D6_SuctOff
        entry: D6A2D2=false; D6SuctOn=false;
        en, du: D6SuctOff = PartStuck80;
      state D6_PartDel
        entry: D6SuctOff=false; D6PartDel=true; D6Transport=false; D6PartStuckM=false;
      state D6_A2M_2
        en, du: D6A2M2 = ~ArmMag80;
      state D6_N4_Wait
        entry: D6A2M2=false;
      state D6_N4_DecCount
        entry: cnt87 = max(cnt87 - 1, 0); D6On = cnt87 > 0;
      state D6_N5_NewCycle
        entry: D6PartDel=false;
      (default) -> OB1_N9_Off
      OB1_N9_Off -> DIST_Ctrl.FB6_Counted.FB6_Wait : [DistInit85 && SimControl_80.SC_85_Counted]
      D6_N5_NewCycle -> DIST_Ctrl.FB6_Counted.FB6_Wait [order 2] : [~D6On]
      DIST_Ctrl.FB6_Counted.FB6_Wait -> FB6_N1_N2_LoadC2 : [(SimSensors_80.SS_81_Start || SimControl_80.SC_85_Start || (CRouteIn80 && KeyPos81)) && ArmMag80 && ElevLow70 && ~PartIn70 && PartinMag80 && cnt80 >= RQ_PARTS]
      FB6_N1_N2_LoadC2 -> D6_A2D_1
      D6_N5_NewCycle -> D6_A2D_1 [order 1] : [D6On]
      D6_A2D_1 -> D6_PistFwd : [ArmDel80 && PistBck80]
      D6_PistFwd -> D6_Transport : [PistFwd80]
      D6_Transport -> D6_A2M_1
      D6_A2M_1 -> D6_SuctOn : [ArmMag80]
      D6_SuctOn -> D6_PartStuck : [PartStuck80]
      D6_PartStuck -> D6_A2D_2
      D6_A2D_2 -> D6_SuctOff : [ArmDel80]
      D6_SuctOff -> D6_PartDel : [~PartStuck80]
      D6_PartDel -> D6_A2M_2
      D6_A2M_2 -> D6_N4_Wait : [ArmMag80]
      D6_N4_Wait -> D6_N4_DecCount [order 1] : [(D6PartDel && TEST_MODE == 1) || (RQPartDel70 && TEST_MODE == 2)]
      D6_N4_Wait -> D6_N5_NewCycle [order 2] : [RQWrong70 && TEST_MODE == 2]
      D6_N4_DecCount -> D6_N5_NewCycle : after(T_DIST_T3,sec)
    state OB1_N10_N11 [parallel]
      settings: executionOrder=3
      state OB1_N10_Wait
      state OB1_N11_PartDel
        entry: PartDel85=true; SimControl_80.SC_85_Part_Del=true; nDistDel = nDistDel + 1;
      state OB1_N10_Hold
        entry: PartDel85=false; SimControl_80.SC_85_Part_Del=false;
      (default) -> OB1_N10_Wait
      OB1_N10_Hold -> OB1_N10_Wait : [~D4PartDel && ~D5PartDelEdge && ~D6PartDel]
      OB1_N10_Wait -> OB1_N11_PartDel : [D4PartDel || D5PartDelEdge || D6PartDel]
      OB1_N11_PartDel -> OB1_N10_Hold : after(T_DIST_T4,sec)
    state FB3_Map80 [parallel]
      settings: executionOrder=7
      state FB3_Map
        during: PistAdv80 = KeyPos81 && (D4PistFwd || D5PistFwd || D6PistFwd);
        SuctOn80 = KeyPos81 && (D4SuctOn || D5SuctOn || D6SuctOn);
        SuctOff80 = KeyPos81 && (D4SuctOff || D5SuctOff || D6SuctOff);
        A2D80 = KeyPos81 && (D4A2D1 || D4A2D2 || D5A2D1 || D5A2D2 || D6A2D1 || D6A2D2);
        A2M80 = KeyPos81 && (FB1A2M2_80 || D4A2M1 || D4A2M2 || D5A2M1 || D5A2M2 || D6A2M1 || D6A2M2);
        SimActuators_80.SA_80_Pist_Adv = PistAdv80; SimActuators_80.SA_80_Suction_On = SuctOn80; SimActuators_80.SA_80_Suction_Off = SuctOff80;
        SimActuators_80.SA_80_Arm_2_Del = A2D80; SimActuators_80.SA_80_Arm_2_Mag = A2M80;
        SimActuators_80.SA_81_Led_Start = KeyPos81 && DistInit85; SimActuators_80.SA_81_Led_Extra1 = PartDel85;
      (default) -> DIST_Ctrl.FB3_Map80.FB3_Map
  state DIST_Plant [parallel]
    entry: KeyPos81=true; magCount = MAG_PARTS0; ArmMag80=true; PistBck80=true;
    MagFull80 = magCount >= MAG_CAP; MagEmpty80 = magCount <= 0;
    SimSensors_80.SS_81_Key_Pos=true; SimSensors_80.SS_81_Start=false; SimSensors_80.SS_81_Stop=false; SimSensors_80.SS_81_Reset=false;
    SimSensors_80.SS_81_Panel_I4=false; SimSensors_80.SS_81_Panel_I5=false; SimSensors_80.SS_81_Panel_I6=false; SimSensors_80.SS_81_Panel_I7=false;
    settings: executionOrder=10
    state Arm [parallel]
      settings: executionOrder=1
      state Arm_AtMag
        entry: ArmMag80=true; ArmDel80=false;
      state Arm_ToDel
        entry: tArm = 0; ArmLoaded = PartInArm;
        during: tArm = tArm + Ts_SIM;
        if ArmLoaded, ArmMag80 = tArm < t_d_magoff_load; else, ArmMag80 = tArm < t_d_magoff_empty; end
      state Arm_AtDel
        entry: ArmDel80=true; ArmMag80=false; SStation70=true;
      state Arm_ToMag
        entry: tArm = 0;
        during: tArm = tArm + Ts_SIM; ArmDel80 = tArm < t_d_deloff;
        if tArm >= t_d_sst_off, SStation70 = false; end
      (default) -> Arm_AtMag
      Arm_ToMag -> Arm_AtMag [order 1] : [tArm >= t_d_a2m]
      Arm_AtMag -> Arm_ToDel : [A2D80 && ~A2M80]
      Arm_ToMag -> Arm_ToDel [order 2] : [A2D80 && ~A2M80]
      Arm_ToDel -> Arm_AtDel [order 1] : [(~ArmLoaded && tArm >= t_d_a2d_empty) || (ArmLoaded && tArm >= t_d_a2d_load)]
      Arm_ToDel -> Arm_ToMag [order 2] : [A2M80 && ~A2D80]
      Arm_AtDel -> Arm_ToMag : [A2M80 && ~A2D80]
    state Suction [parallel]
      settings: executionOrder=3
      state Suct_Idle
      state Suct_Gripping
      state Suct_Holding
        entry: PartStuck80=true; PartInArm=true; PartAtPickup=false;
      state Suct_Release
      state Suct_Dropped
        entry: PartStuck80=false; PartInArm=false;
        if ArmDel80, PartIn70 = true; testColor = PART_COLORS(min(nTestIn + 1, numel(PART_COLORS))); nTestIn = nTestIn + 1; SInd70 = (testColor == 3); end
      (default) -> Suct_Idle
      Suct_Dropped -> Suct_Idle
      Suct_Idle -> Suct_Gripping : [SuctOn80 && ArmMag80 && PartAtPickup]
      Suct_Gripping -> Suct_Holding : after(t_d_suct,sec)
      Suct_Holding -> Suct_Release : [~SuctOn80]
      Suct_Release -> Suct_Dropped : after(t_d_release,sec)
    state MagPiston [parallel]
      settings: executionOrder=2
      state DPist_Back
        entry: PistBck80=true; PistFwd80=false;
      state DPist_Fwd
        entry: tPistD = 0;
        during: tPistD = tPistD + Ts_SIM; PistBck80 = tPistD < t_d_pist_bckoff;
        if tPistD >= t_d_pist_fwd && ~PistFwd80
        PistFwd80 = true;
        if magCount > 0, magCount = magCount - 1; PartAtPickup = true; end
        end
      state DPist_Return
        entry: PistFwd80=false;
      (default) -> DPist_Back
      DPist_Return -> DPist_Back : after(t_d_pist_back,sec)
      DPist_Back -> DPist_Fwd : [PistAdv80]
      DPist_Fwd -> DPist_Return : [~PistAdv80]
    state Sensors_Out80 [parallel]
      settings: executionOrder=4
      state S80_Map
        en, du: MagFull80 = magCount >= MAG_CAP; MagEmpty80 = magCount <= 0;
        SimSensors_80.SS_80_Arm_Mag = ArmMag80; SimSensors_80.SS_80_Arm_Del = ArmDel80; SimSensors_80.SS_80_Pist_Bck = PistBck80;
        SimSensors_80.SS_80_Pist_Fwd = PistFwd80; SimSensors_80.SS_80_Part_Stuck = PartStuck80;
        SimSensors_80.SS_80_Mag_Full = MagFull80; SimSensors_80.SS_80_Mag_Empty = MagEmpty80;
      (default) -> S80_Map
  state PROC_Ctrl [parallel]
    entry: SimControl_100.SC_102_Profibus=false; SimControl_100.SC_103_RQ_Turns = RQ_TURNS; SimControl_100.SC_105_Initialization=false; SimControl_100.SC_105_Start=false;
    SimControl_100.SC_105_Part_ready=false; SimControl_100.SC_105_Test_Ok=false; SimControl_100.SC_105_Test_Fail=false; SimControl_100.SC_106_RT_Counter=0;
    SimControl_100.SC_105_Test = (PROC_MODE == 1); SimControl_100.SC_105_TestDrill = (PROC_MODE == 2); SimControl_100.SC_105_Rotation = (PROC_MODE == 3);
    SimActuators_100.SA_100_Drill_On=false; SimActuators_100.SA_100_RT_On=false; SimActuators_100.SA_100_Drill_Down=false; SimActuators_100.SA_100_Drill_Up=false; SimActuators_100.SA_100_Drill_Pin=false; SimActuators_100.SA_100_Test_Pin=false; SimActuators_100.SA_101_Led_Start=false; SimActuators_100.SA_101_Led_Reset=false; SimActuators_100.SA_101_Led_Extra1=false; SimActuators_100.SA_101_Led_Extra2=false; SimActuators_100.SA_101_Panel_O4=false; SimActuators_100.SA_101_Panel_O5=false; SimActuators_100.SA_101_Panel_O6=false; SimActuators_100.SA_101_Panel_O7=false;
    settings: executionOrder=11
    state FB1_Init100 [parallel]
      settings: executionOrder=1
      state FB1_N2_DrillUp
        entry: SimControl_100.SC_102_Profibus=true; ProcInit=false;
        en, du: P1DrillUp = ~SDrillHigh100;
      state FB1_N3_Empty1
        entry: P1DrillUp=false; P1DrillH=true;
      state FB1_N4_Rotate3
        entry: P1Empty1=true; cntRT = 3; P1RT1=true;
      state FB1_N5_Empty2
        entry: P1RT1=false;
      state FB1_N12_InitOk
        entry: P1Empty2=true; ProcInit=true; SimControl_100.SC_105_Initialization=true;
      state FB1_N6_N11_Clear
        entry: ProcInit=false;
      (default) -> FB1_N2_DrillUp
      FB1_N2_DrillUp -> FB1_N3_Empty1 : [SDrillHigh100]
      FB1_N3_Empty1 -> FB1_N4_Rotate3 [order 1] : [~RtOn100 && RTSens100 && ~PInit100 && ~PDrill100 && ~PTest100]
      FB1_N3_Empty1 -> FB1_N6_N11_Clear [order 2] : [~RtOn100 && RTSens100 && (PInit100 || PDrill100 || PTest100)]
      FB1_N4_Rotate3 -> FB1_N5_Empty2 : [cntRT <= 0]
      FB1_N5_Empty2 -> FB1_N12_InitOk [order 1] : [~RtOn100 && RTSens100 && ~PInit100 && ~PDrill100 && ~PTest100]
      FB1_N5_Empty2 -> FB1_N6_N11_Clear [order 2] : [~RtOn100 && RTSens100 && (PInit100 || PDrill100 || PTest100)]
    state OB1_N4_N8 [parallel]
      settings: executionOrder=2
      state OB1_N4_N8_Map
        en, du: PartReady100 = P4Ready || P5Ready || P6Ready; SimControl_100.SC_105_Part_ready = PartReady100;
        if RtOn100 && RTSens100 && ~prevRTSens100, cnt106 = cnt106 + 1; end
        if ~RtOn100, cnt106 = 0; end
        if RTSens100 && ~prevRTSens100 && cntRT > 0, cntRT = cntRT - 1; end
        prevRTSens100 = RTSens100; SimControl_100.SC_106_RT_Counter = cnt106;
      (default) -> OB1_N4_N8_Map
    state FB4_Test [parallel]
      settings: executionOrder=3
      state OB1_N5_Off
      state FB4_Wait
      state FB4_N1_StartTest
        entry: P4Start=true; SimControl_100.SC_105_Test_Ok=false; SimControl_100.SC_105_Test_Fail=false; P4OK=false; P4Fail=false;
      state FB4_N2_SpinToTest
        entry: cntRT = 4; P4RT=true;
      state FB4_N3_T4_TestDelay
        entry: P4RT=false;
      state FB4_N4_TestPin
        entry: P4Pin=true;
      state FB4_N5_N6_Result
        entry: P4OK = PTestOk100; P4Fail = ~PTestOk100;
        SimControl_100.SC_105_Test_Ok = P4OK; SimControl_100.SC_105_Test_Fail = P4Fail;
      state FB4_N7_SpinToCollect
        entry: P4Pin=false; cntRT = 2; P4RT=true;
      state FB4_N8_PartReady
        entry: P4RT=false; P4Ready=true;
      state FB4_N9_PickedUp
        entry: P4Ready=false; P4OK=false; P4Fail=false; P4Start=false;
      (default) -> PROC_Ctrl.FB4_Test.OB1_N5_Off
      PROC_Ctrl.FB4_Test.OB1_N5_Off -> PROC_Ctrl.FB4_Test.FB4_Wait : [ProcInit && SimControl_100.SC_105_Test]
      FB4_N9_PickedUp -> PROC_Ctrl.FB4_Test.FB4_Wait
      PROC_Ctrl.FB4_Test.FB4_Wait -> FB4_N1_StartTest : [PInit100 && ClawHigh90 && RTSens100 && ~RtOn100]
      FB4_N1_StartTest -> FB4_N2_SpinToTest
      FB4_N2_SpinToTest -> FB4_N3_T4_TestDelay : [cntRT <= 0]
      FB4_N3_T4_TestDelay -> FB4_N4_TestPin : [~RtOn100 && PTest100 && RTSens100]
      FB4_N4_TestPin -> FB4_N5_N6_Result : after(T_PROC_T5,sec)
      FB4_N5_N6_Result -> FB4_N7_SpinToCollect
      FB4_N7_SpinToCollect -> FB4_N8_PartReady : [cntRT <= 0]
      FB4_N8_PartReady -> FB4_N9_PickedUp : [ClawDel90 && ClawLow90 && PartInClaw90]
    state FB5_TestDrill [parallel]
      settings: executionOrder=4
      state OB1_N6_Off
      state FB5_Wait
      state FB5_N1_StartTD
        entry: P5Start=true; SimControl_100.SC_105_Test_Ok=false; SimControl_100.SC_105_Test_Fail=false; P5OK=false; P5Fail=false; P5DrillOk=false;
      state FB5_N2_SpinToTest
        entry: cntRT = 4; P5RT=true;
      state FB5_N3_T4_TestDelay
        entry: P5RT=false;
      state FB5_N4_TestPin
        entry: P5Pin=true;
      state FB5_N5_N6_Result
        entry: P5OK = PTestOk100; P5Fail = ~PTestOk100;
        SimControl_100.SC_105_Test_Ok = P5OK; SimControl_100.SC_105_Test_Fail = P5Fail;
      state FB5_N7_SpinToDrill
        entry: P5Pin=false; cntRT = 1; P5RT=true;
      state FB5_N8_PinLowerDrill
        entry: P5RT=false; P5DrillPin=true; P5LDrill=true;
      state FB5_N9_N10_T8_Drill
        entry: P5TDrill=true;
      state FB5_N11_RaiseDrill
        entry: P5TDrill=false; P5LDrill=false; P5RDrill=true;
      state FB5_N12_N13_SpinFinal
        entry: P5DrillPin=false; P5RDrill=false; P5DrillOk=true; cntRT = 1; P5RT=true;
      state FB5_N14_SpinFinalFail
        entry: P5Pin=false; cntRT = 2; P5RT=true;
      state FB5_N15_PartReady
        entry: P5RT=false; P5Ready=true;
      state FB5_N16_PickedUp
        entry: P5Ready=false; P5OK=false; P5Fail=false; P5DrillOk=false; P5Start=false;
      (default) -> OB1_N6_Off
      OB1_N6_Off -> PROC_Ctrl.FB5_TestDrill.FB5_Wait : [ProcInit && SimControl_100.SC_105_TestDrill]
      FB5_N16_PickedUp -> PROC_Ctrl.FB5_TestDrill.FB5_Wait
      PROC_Ctrl.FB5_TestDrill.FB5_Wait -> FB5_N1_StartTD : [PInit100 && ClawHigh90 && RTSens100 && ~RtOn100]
      FB5_N1_StartTD -> FB5_N2_SpinToTest
      FB5_N2_SpinToTest -> FB5_N3_T4_TestDelay : [cntRT <= 0]
      FB5_N3_T4_TestDelay -> FB5_N4_TestPin : [~RtOn100 && PTest100 && RTSens100]
      FB5_N4_TestPin -> FB5_N5_N6_Result : after(T_PROC_T5,sec)
      FB5_N5_N6_Result -> FB5_N7_SpinToDrill [order 1] : [P5OK]
      FB5_N5_N6_Result -> FB5_N14_SpinFinalFail [order 2] : [P5Fail]
      FB5_N7_SpinToDrill -> FB5_N8_PinLowerDrill : [cntRT <= 0]
      FB5_N8_PinLowerDrill -> FB5_N9_N10_T8_Drill : [SDrillLow100]
      FB5_N9_N10_T8_Drill -> FB5_N11_RaiseDrill : after(T_PROC_T8,sec)
      FB5_N11_RaiseDrill -> FB5_N12_N13_SpinFinal : [SDrillHigh100]
      FB5_N12_N13_SpinFinal -> FB5_N15_PartReady : [cntRT <= 0]
      FB5_N14_SpinFinalFail -> FB5_N15_PartReady : [cntRT <= 0]
      FB5_N15_PartReady -> FB5_N16_PickedUp : [ClawDel90 && ClawLow90 && PartInClaw90]
    state FB6_Rotation [parallel]
      settings: executionOrder=5
      state OB1_N7_Off
      state FB6_Wait
      state FB6_N1_StartR
        entry: P6Start=true; P6RotOK=false;
      state FB6_N2_Spin6
        entry: cntRT = 6; P6RT=true;
      state FB6_N3_N4_RotationOK
        entry: P6RT=false; P6RotOK=true; P6Ready=true;
      state FB6_N5_PickedUp
        entry: P6Ready=false; P6RotOK=false; P6Start=false;
      (default) -> PROC_Ctrl.FB6_Rotation.OB1_N7_Off
      PROC_Ctrl.FB6_Rotation.OB1_N7_Off -> PROC_Ctrl.FB6_Rotation.FB6_Wait : [ProcInit && SimControl_100.SC_105_Rotation]
      FB6_N5_PickedUp -> PROC_Ctrl.FB6_Rotation.FB6_Wait
      PROC_Ctrl.FB6_Rotation.FB6_Wait -> FB6_N1_StartR : [PInit100 && ClawHigh90 && ~RtOn100]
      FB6_N1_StartR -> FB6_N2_Spin6
      FB6_N2_Spin6 -> FB6_N3_N4_RotationOK : [cntRT <= 0]
      FB6_N3_N4_RotationOK -> FB6_N5_PickedUp : [ClawDel90 && ClawLow90 && PartInClaw90]
    state FB3_Map100 [parallel]
      settings: executionOrder=6
      state FB3_Map
        during: RtOn100 = KeyPos101 && ((P1RT1 && cntRT > 0 && (ClawHigh90 || ~ClawDel90)) || (P4RT && cntRT > 0) || (P5RT && cntRT > 0) || (P6RT && cntRT > 0));
        DrillDown100 = KeyPos101 && P5LDrill; DrillUp100 = KeyPos101 && (P1DrillUp || P5RDrill);
        DrillPin100 = KeyPos101 && P5DrillPin; DrillOn100 = KeyPos101 && P5TDrill; TestPin100 = KeyPos101 && (P4Pin || P5Pin);
        SimActuators_100.SA_100_RT_On = RtOn100; SimActuators_100.SA_100_Drill_Down = DrillDown100; SimActuators_100.SA_100_Drill_Up = DrillUp100;
        SimActuators_100.SA_100_Drill_Pin = DrillPin100; SimActuators_100.SA_100_Drill_On = DrillOn100; SimActuators_100.SA_100_Test_Pin = TestPin100;
        SimActuators_100.SA_101_Led_Start = KeyPos101 && ProcInit; SimActuators_100.SA_101_Led_Extra1 = PartReady100;
      (default) -> PROC_Ctrl.FB3_Map100.FB3_Map
  state PROC_Plant [parallel]
    entry: KeyPos101=true; RTSens100=true; SDrillHigh100=true;
    SimSensors_100.SS_101_Key_Pos=true; SimSensors_100.SS_101_Start=false; SimSensors_100.SS_101_Stop=false; SimSensors_100.SS_101_Reset=false;
    SimSensors_100.SS_101_Panel_I4=false; SimSensors_100.SS_101_Panel_I5=false; SimSensors_100.SS_101_Panel_I6=false; SimSensors_100.SS_101_Panel_I7=false;
    settings: executionOrder=12
    state Table [parallel]
      settings: executionOrder=1
      state RT_Stopped
      state RT_Moving
        entry: tRt = 0;
        during: tRt = tRt + Ts_SIM;
        if tRt >= t_rt_step, tRt = 0; RTSens100 = true; partOff = mod(partOff + 1, 6);
        elseif tRt >= t_rt_hi, RTSens100 = false; end
      (default) -> RT_Stopped
      RT_Moving -> RT_Stopped : [~RtOn100]
      RT_Stopped -> RT_Moving : [RtOn100]
    state Probe_Sensors [parallel]
      settings: executionOrder=3
      state Sens_Map
        en, du: PInit100 = PartOnTable && partOff == 0 && ~RtOn100;
        PTest100 = PartOnTable && partOff == 4 && ~RtOn100; PDrill100 = PartOnTable && partOff == 5 && ~RtOn100;
        SimSensors_100.SS_100_PInit_Pos = PInit100; SimSensors_100.SS_100_PTest_Pos = PTest100; SimSensors_100.SS_100_PDrill_Pos = PDrill100;
        SimSensors_100.SS_100_RT_Sensor = RTSens100; SimSensors_100.SS_100_SDrill_High = SDrillHigh100; SimSensors_100.SS_100_SDrill_Low = SDrillLow100;
        SimSensors_100.SS_100_PTest_Ok = PTestOk100;
      (default) -> PROC_Plant.Probe_Sensors.Sens_Map
    state Drill [parallel]
      settings: executionOrder=2
      state Drill_Up
        entry: SDrillHigh100=true; SDrillLow100=false;
      state Drill_GoingDown
        entry: SDrillHigh100=false;
      state Drill_Low
        entry: SDrillLow100=true;
      state Drill_GoingUp
        entry: SDrillLow100=false;
      (default) -> Drill_Up
      Drill_GoingUp -> Drill_Up : after(t_drill_up,sec)
      Drill_Up -> Drill_GoingDown : [DrillDown100 && ~DrillUp100]
      Drill_GoingDown -> Drill_Low : after(t_drill_down,sec)
      Drill_Low -> Drill_GoingUp : [DrillUp100]
    state TestProbe [parallel]
      settings: executionOrder=4
      state Probe_Up
        entry: PTestOk100=false;
      state Probe_Down
      state Probe_Read
        entry: PTestOk100 = PTest100 && PROC_TEST_OK(min(max(procIdx,1), numel(PROC_TEST_OK))) == 1;
      (default) -> Probe_Up
      Probe_Read -> Probe_Up : [~TestPin100]
      Probe_Up -> Probe_Down : [TestPin100]
      Probe_Down -> Probe_Read : after(t_ptest_ok,sec)
  state HD2_Ctrl [parallel]
    entry: SimControl_90.SC_92_Profibus=false; SimControl_90.SC_95_Initialization=false; SimControl_90.SC_95_Start=false; SimControl_90.SC_95_PD_Proc=false; SimControl_90.SC_95_PD_Cart=false;
    SimControl_90.SC_95_Cart2Del = (HD2_CART2DEL == 1); SimControl_90.SC_95_Del2Cart = (HD2_DEL2CART == 1);
    SimASi_90.SR_93_ProcCartID=0; SimASi_90.SR_94_Request=false; SimASi_90.SR_94_No_Cart=true; SimASi_90.SR_94_Cart_Full=false; SimASi_90.SR_94_CRoute_Out=false; SimASi_90.SR_94_CRoute_In=false;
    SimActuators_90.SA_90_Claw_2_Cart=false; SimActuators_90.SA_90_Claw_2_Del=false; SimActuators_90.SA_90_Claw_Down=false; SimActuators_90.SA_90_Close_Claw=false; SimActuators_90.SA_91_Led_Start=false; SimActuators_90.SA_91_Led_Reset=false; SimActuators_90.SA_91_Led_Extra1=false; SimActuators_90.SA_91_Led_Extra2=false; SimActuators_90.SA_91_Panel_O4=false; SimActuators_90.SA_91_Panel_O5=false; SimActuators_90.SA_91_Panel_O6=false; SimActuators_90.SA_91_Panel_O7=false;
    settings: executionOrder=13
    state FB1_Init90 [parallel]
      settings: executionOrder=1
      state FB1_N2_N3_Check
        entry: SimControl_90.SC_92_Profibus=true; H2Init=false; SimControl_90.SC_95_Initialization=false;
        during: H2Arm2Cart = ClawHigh90 && ~ClawCart90; H2ClawHighC = ~ClawHigh90;
      state FB1_N4_N5_Deliver
        entry: H2Arm2Cart=false;
      state FB1_N1_N2_InitOk
        entry: H2Arm2Cart=false; H2ClawHighC=false; H2Init=true; SimControl_90.SC_95_Initialization=true;
      (default) -> HD2_Ctrl.FB1_Init90.FB1_N2_N3_Check
      HD2_Ctrl.FB1_Init90.FB1_N2_N3_Check -> FB1_N1_N2_InitOk [order 1] : [ClawHigh90 && ~PartInClaw90 && ClawCart90]
      HD2_Ctrl.FB1_Init90.FB1_N2_N3_Check -> FB1_N4_N5_Deliver [order 2] : [PartInClaw90]
    state OB1_N4_N7_N9 [parallel]
      settings: executionOrder=2
      state OB1_Map90
        en, du: OKMove90 = CartStat25 && ~PartInClaw90 && ((HD2_CART2DEL == 1 && ~PInit100) || (HD2_DEL2CART == 1 && ~Optic25));
        SimControl_90.SC_95_PD_Proc = H4PartDel; SimControl_90.SC_95_PD_Cart = H5PartDel; SimASi_90.SR_94_No_Cart = ~CartStat25;
        SimASi_90.SR_94_CRoute_In = CRouteIn94; SimASi_90.SR_94_Cart_Full = CartStat25 && Optic25;
      (default) -> OB1_Map90
    state FB4_Cart2Del [parallel]
      settings: executionOrder=4
      state FB4_Wait
      state FB4_N1_Begin
        entry: H4P2D=true; H4PartDel=false; H5PartDel=false;
      state FB4_N2_ArmToCart
        en, du: H4Claw2Cart = ~ClawCart90;
      state FB4_N2_ProcStart
        entry: H4Claw2Cart=false; H4ProcStart=true;
      state FB4_N3_Lower
        entry: H4Low1=true;
      state FB4_N3_Close
        entry: H4Close=true;
      state FB4_N3_Raise
        entry: H4Low1=false;
      state FB4_N4_Claw2Del
        en, du: H4Claw2Del = ~ClawDel90;
      state FB4_N5_Lower2
        entry: H4Claw2Del=false; H4Low2=true;
      state FB4_N5_Open
        entry: H4Close=false;
      state FB4_N5_Raise
        entry: H4Low2=false;
      state FB4_N6_PartDelivered
        entry: H4PartDel=true; H4P2D=false; H4ProcStart=false;
      (default) -> HD2_Ctrl.FB4_Cart2Del.FB4_Wait
      FB4_N6_PartDelivered -> HD2_Ctrl.FB4_Cart2Del.FB4_Wait
      HD2_Ctrl.FB4_Cart2Del.FB4_Wait -> FB4_N1_Begin : [H2Init && ((OKMove90 && HD2_CART2DEL == 1) || H4P2D) && CRouteIn94 && KeyPos91]
      FB4_N1_Begin -> FB4_N2_ArmToCart
      FB4_N2_ArmToCart -> FB4_N2_ProcStart : [ClawCart90]
      FB4_N2_ProcStart -> FB4_N3_Lower : [ClawCart90 && ~ClawLow90 && ~PartInClaw90]
      FB4_N3_Lower -> FB4_N3_Close : [ClawLow90]
      FB4_N3_Close -> FB4_N3_Raise : [PartInClaw90]
      FB4_N3_Raise -> FB4_N4_Claw2Del : [ClawHigh90 && PartInClaw90]
      FB4_N4_Claw2Del -> FB4_N5_Lower2 : [ClawDel90 && ClawHigh90 && PartInClaw90]
      FB4_N5_Lower2 -> FB4_N5_Open : [ClawLow90]
      FB4_N5_Open -> FB4_N5_Raise : [~CloseClaw90]
      FB4_N5_Raise -> FB4_N6_PartDelivered : [ClawDel90 && ClawHigh90 && ~PartInClaw90]
    state FB5_Del2Cart [parallel]
      settings: executionOrder=5
      state FB5_Wait
      state FB5_N1_Begin
        entry: H5P2D=true; H5PartDel=false; H4PartDel=false;
      state FB5_N2_ArmToDel
        en, du: H5Claw2Del = ~ClawDel90;
      state FB5_N2_ProcStart
        entry: H5Claw2Del=false; H5ProcStart=true;
      state FB5_N3_Lower
        entry: H5Low1=true;
      state FB5_N3_Close
        entry: H5Close=true;
      state FB5_N3_Raise
        entry: H5Low1=false;
      state FB5_N4_Claw2Cart
        en, du: H5Claw2Cart = ~ClawCart90;
      state FB5_N5_Lower2
        entry: H5Claw2Cart=false; H5Low2=true;
      state FB5_N5_Open
        entry: H5Close=false;
      state FB5_N5_Raise
        entry: H5Low2=false;
      state FB5_N6_PartDelivered
        entry: H5PartDel=true; H5P2D=false; H5ProcStart=false;
      (default) -> HD2_Ctrl.FB5_Del2Cart.FB5_Wait
      FB5_N6_PartDelivered -> HD2_Ctrl.FB5_Del2Cart.FB5_Wait
      HD2_Ctrl.FB5_Del2Cart.FB5_Wait -> FB5_N1_Begin : [H2Init && ((OKMove90 && HD2_DEL2CART == 1) || (PartReady100 && ~Optic25)) && (PartReady100 || SimControl_90.SC_95_Start)]
      FB5_N1_Begin -> FB5_N2_ArmToDel
      FB5_N2_ArmToDel -> FB5_N2_ProcStart : [ClawDel90]
      FB5_N2_ProcStart -> FB5_N3_Lower : [ClawDel90 && ~ClawLow90 && ~PartInClaw90]
      FB5_N3_Lower -> FB5_N3_Close : [ClawLow90]
      FB5_N3_Close -> FB5_N3_Raise : [PartInClaw90]
      FB5_N3_Raise -> FB5_N4_Claw2Cart : [ClawHigh90 && PartInClaw90]
      FB5_N4_Claw2Cart -> FB5_N5_Lower2 : [ClawCart90 && ClawHigh90 && PartInClaw90]
      FB5_N5_Lower2 -> FB5_N5_Open : [ClawLow90]
      FB5_N5_Open -> FB5_N5_Raise : [~CloseClaw90]
      FB5_N5_Raise -> FB5_N6_PartDelivered : [ClawCart90 && ClawHigh90 && ~PartInClaw90]
    state OB1_N8_T1_CRouteOut [parallel]
      settings: executionOrder=3
      state OB1_N8_Wait
      state OB1_N8_Pulse
        entry: RouteOut94=true; SimASi_90.SR_94_CRoute_Out=true;
      state OB1_N8_Hold
        entry: RouteOut94=false; SimASi_90.SR_94_CRoute_Out=false;
      (default) -> OB1_N8_Wait
      OB1_N8_Hold -> OB1_N8_Wait : [~H5PartDel]
      OB1_N8_Wait -> OB1_N8_Pulse : [H5PartDel]
      OB1_N8_Pulse -> OB1_N8_Hold [order 1] : after(T_HD2_T1,sec)
      OB1_N8_Pulse -> OB1_N8_Hold [order 2] : [~H5PartDel]
    state FB3_Map90 [parallel]
      settings: executionOrder=6
      state FB3_Map
        during: Claw2Cart90 = KeyPos91 && (H2Arm2Cart || H4Claw2Cart || H5Claw2Cart);
        Claw2Del90 = KeyPos91 && (H4Claw2Del || H5Claw2Del);
        ClawDown90 = KeyPos91 && (H4Low1 || H4Low2 || H5Low1 || H5Low2);
        CloseClaw90 = KeyPos91 && (H4Close || H5Close);
        SimActuators_90.SA_90_Claw_2_Cart = Claw2Cart90; SimActuators_90.SA_90_Claw_2_Del = Claw2Del90; SimActuators_90.SA_90_Claw_Down = ClawDown90; SimActuators_90.SA_90_Close_Claw = CloseClaw90;
        SimActuators_90.SA_91_Led_Start = KeyPos91 && H2Init; SimActuators_90.SA_91_Led_Extra1 = H5PartDel;
      (default) -> HD2_Ctrl.FB3_Map90.FB3_Map
  state HD2_Plant [parallel]
    entry: KeyPos91=true; ClawHigh90=true; ClawCart90=true;
    SimSensors_90.SS_91_Key_Pos=true; SimSensors_90.SS_91_Start=false; SimSensors_90.SS_91_Stop=true; SimSensors_90.SS_91_Reset=false; SimSensors_90.SS_90_Part_Reserve=false;
    SimSensors_90.SS_91_Panel_I4=false; SimSensors_90.SS_91_Panel_I5=false; SimSensors_90.SS_91_Panel_I6=false; SimSensors_90.SS_91_Panel_I7=false;
    settings: executionOrder=14
    state Vertical [parallel]
      settings: executionOrder=1
      state V_High
        entry: ClawHigh90=true; ClawLow90=false;
      state V_GoingDown
        entry: tC2v = 0;
        during: tC2v = tC2v + Ts_SIM; ClawHigh90 = tC2v < t_c2_highoff;
      state V_Low
        entry: ClawLow90=true; ClawHigh90=false;
      state V_GoingUp
        entry: tC2v = 0;
        during: tC2v = tC2v + Ts_SIM; ClawLow90 = tC2v < t_c2_lowoff;
      (default) -> V_High
      V_GoingUp -> V_High [order 1] : [tC2v >= t_c2_up]
      V_High -> V_GoingDown : [ClawDown90]
      V_GoingUp -> V_GoingDown [order 2] : [ClawDown90]
      V_GoingDown -> V_Low [order 1] : [tC2v >= t_c2_down]
      V_GoingDown -> V_GoingUp [order 2] : [~ClawDown90]
      V_Low -> V_GoingUp : [~ClawDown90]
    state Horizontal [parallel]
      settings: executionOrder=2
      state H_AtCart
        entry: ClawCart90=true; ClawDel90=false;
      state H_ToDel
        entry: tC2h = 0;
        during: tC2h = tC2h + Ts_SIM; ClawCart90 = tC2h < t_c2_cartoff;
      state H_AtDel
        entry: ClawDel90=true; ClawCart90=false;
      state H_ToCart
        entry: tC2h = 0;
        during: tC2h = tC2h + Ts_SIM; ClawDel90 = tC2h < t_c2_deloff;
      (default) -> H_AtCart
      H_ToCart -> H_AtCart : [tC2h >= t_c2_2cart]
      H_AtCart -> H_ToDel : [Claw2Del90 && ~Claw2Cart90]
      H_ToDel -> H_AtDel : [tC2h >= t_c2_2del]
      H_AtDel -> H_ToCart : [Claw2Cart90 && ~Claw2Del90]
    state Gripper [parallel]
      settings: executionOrder=3
      state G_Open
        entry: PartInClaw90=false;
      state G_Closing
      state G_Holding
        entry: PartInClaw90=true;
        if ClawDel90, PartOnTable=false; else, cartPart=false; end
      state G_Opening
      state G_Released
        entry: PartInClaw90=false;
        if ClawDel90, PartOnTable=true; partOff=0; nProcIn = nProcIn + 1; procIdx = nProcIn;
        else, cartPart=true; end
      (default) -> G_Open
      G_Released -> G_Open
      G_Open -> G_Closing : [CloseClaw90 && ClawLow90 && ((ClawDel90 && PartOnTable) || (ClawCart90 && CartHasPart25))]
      G_Closing -> G_Holding : after(t_c2_grip,sec)
      G_Holding -> G_Opening : [~CloseClaw90]
      G_Opening -> G_Released : after(t_c2_open,sec)
    state Sensors_Out90 [parallel]
      settings: executionOrder=4
      state S90_Map
        en, du: SimSensors_90.SS_90_Claw_High = ClawHigh90; SimSensors_90.SS_90_Claw_Low = ClawLow90; SimSensors_90.SS_90_Claw_Del = ClawDel90;
        SimSensors_90.SS_90_Claw_Cart = ClawCart90; SimSensors_90.SS_90_Part_in_Claw = PartInClaw90;
        SimSensors_90.SS_90_Claw_Reserve = (Claw2Del90 && tC2h >= t_c2_res_del && tC2h < t_c2_res_del + t_c2_res_dur) || (Claw2Cart90 && tC2h >= t_c2_res_cart && tC2h < t_c2_res_cart + t_c2_res_dur);
      (default) -> S90_Map
  state ROB_Ctrl [parallel]
    entry: SimControl_30.SC_30_Robot1 = (ROBOT_MODE == 1); SimControl_30.SC_30_Robot2 = (ROBOT_MODE == 2); SimControl_30.SC_35_Part_Del=false;
    SimASi_30.SR_32_RoboCartID=0; SimASi_30.SR_34_Request=false; SimASi_30.SR_34_No_Cart=true; SimASi_30.SR_34_Cart_Full=false; SimASi_30.SR_34_CRoute_Out=false; SimASi_30.SR_34_CRoute_In=false;
    SimActuators_30.SA_30_Led_Start=false; SimActuators_30.SA_30_Led_Reset=false; SimActuators_30.SA_30_Spring_Cyl=false; SimActuators_30.SA_30_Cover_Cyl=false;
    SimRFID_RFID.SID_Ant1_R_TagID=0; SimRFID_RFID.SID_Ant1_R_UserData=0; SimRFID_RFID.SID_Ant1_W_TagID=0; SimRFID_RFID.SID_Ant1_W_UserData=0;
    SimRFID_RFID.SID_Ant2_R_TagID=0; SimRFID_RFID.SID_Ant2_R_UserData=0; SimRFID_RFID.SID_Ant2_W_TagID=0; SimRFID_RFID.SID_Ant2_W_UserData=0;
    SimRFID_RFID.SID_Ant3_R_TagID=0; SimRFID_RFID.SID_Ant3_R_UserData=0; SimRFID_RFID.SID_Ant3_W_TagID=0; SimRFID_RFID.SID_Ant3_W_UserData=0;
    SimRFID_RFID.SID_Ant4_R_TagID=0; SimRFID_RFID.SID_Ant4_R_UserData=0; SimRFID_RFID.SID_Ant4_W_TagID=0; SimRFID_RFID.SID_Ant4_W_UserData=0;
    settings: executionOrder=15
    state FB3_N4_N11_Map [parallel]
      settings: executionOrder=1
      state FB3_Map30
        en, du: SimASi_30.SR_34_No_Cart = ~CartStat27; SimASi_30.SR_34_Cart_Full = CartStat27 && Optic27; SimASi_30.SR_34_CRoute_In = CRouteIn34;
        SimActuators_30.SA_30_Led_Extra1 = ~CartStat27; SimActuators_30.SA_30_Led_Extra2 = CartStat27 && Optic27;
      (default) -> FB3_Map30
    state FB3_N12_N14_Route [parallel]
      settings: executionOrder=2
      state N12_Wait
      state N12_T7_CartDel
        entry: RobCartDel=true;
      state N13_PartDel
        entry: RobCartDel=false; PartDel35=true; RouteOut34=true; SimControl_30.SC_35_Part_Del=true; SimASi_30.SR_34_CRoute_Out=true;
      state N14_T8_Reset
        entry: PartDel35=false; RouteOut34=false; SimControl_30.SC_35_Part_Del=false; SimASi_30.SR_34_CRoute_Out=false;
      (default) -> N12_Wait
      N14_T8_Reset -> N12_Wait : [~CRouteIn34]
      N12_Wait -> N12_T7_CartDel : [CRouteIn34 && (ROBOT_MODE == 1 || ROBOT_MODE == 2)]
      N12_T7_CartDel -> N13_PartDel [order 1] : [~CRouteIn34]
      N12_T7_CartDel -> N13_PartDel [order 2] : after(T_ROB_T7,sec)
      N13_PartDel -> N14_T8_Reset : after(T_ROB_T8,sec)
  state ROB_Plant [parallel]
    entry: SimSensors_30.SS_31_Start=false; SimSensors_30.SS_31_Stop=true; SimSensors_30.SS_31_Reset=false; SimSensors_30.SS_31_Part_in_Claw=false; SimSensors_30.SS_31_Orientation=false;
    SimSensors_30.SS_32_Sp_Cyl_Bck=true; SimSensors_30.SS_32_Sp_Cyl_Fwd=false; SimSensors_30.SS_32_Co_Cyl_Bck=true; SimSensors_30.SS_32_Co_Cyl_Fwd=false;
    SimSensors_30.SS_32_Sp_PickUp=true; SimSensors_30.SS_32_Co_PickUp=false; SimSensors_30.SS_32_CoMag_Empty=false;
    settings: executionOrder=17
    state ROB_Rest
    (default) -> ROB_Rest
  state STOR_Ctrl [parallel]
    entry: SimControl_40.SC_42_Profibus=false; SimControl_40.SC_45_Initialization=false; SimControl_40.SC_45_Start=false;
    SimControl_40.SC_45_StorePart = (STOR_MODE == 1); SimControl_40.SC_45_RetrievePart = (STOR_MODE == 2);
    SimASi_40.SR_43_StorCartID=0; SimASi_40.SR_44_Request=false; SimASi_40.SR_44_No_Cart=true; SimASi_40.SR_44_Cart_Full=false; SimASi_40.SR_44_CRoute_Out=false; SimASi_40.SR_44_CRoute_In=false;
    SimActuators_40.SA_41_Led_Reset=false; SimActuators_40.SA_41_Panel_O4=false; SimActuators_40.SA_41_Panel_O5=false; SimActuators_40.SA_41_Panel_O6=false; SimActuators_40.SA_41_Panel_O7=false;
    settings: executionOrder=18
    state FB1_Init40 [parallel]
      settings: executionOrder=1
      state FB1_N1_Profibus
        entry: SimControl_40.SC_42_Profibus=true; StorInit=false;
      state FB1_N1_InitOk
        entry: StorInit=true; SimControl_40.SC_45_Initialization=true;
      (default) -> FB1_N1_Profibus
      FB1_N1_Profibus -> STOR_Ctrl.FB1_Init40.FB1_N1_InitOk
    state FB4_Store [parallel]
      settings: executionOrder=2
      state OB1_N4_Wait
      state N1_T1_SPEXT
        entry: StoreOK=true; ProcessOK44=false;
      state OB1_N6_NEG_ProcOK
        entry: StoreOK=false; ProcessOK44=true;
      (default) -> OB1_N4_Wait
      STOR_Ctrl.FB4_Store.OB1_N6_NEG_ProcOK -> OB1_N4_Wait : [~CRouteIn44]
      OB1_N4_Wait -> N1_T1_SPEXT : [StorInit && STOR_MODE == 1 && CRouteIn44 && KeyPos41]
      N1_T1_SPEXT -> STOR_Ctrl.FB4_Store.OB1_N6_NEG_ProcOK : after(T_STOR_T1,sec)
    state FB5_Retrieve [parallel]
      settings: executionOrder=3
      state OB1_N5_Wait
      state N1_T2_SPEXT
        entry: RetrieveOK=true; ProcessOK44=false;
      state OB1_N6_NEG_ProcOK
        entry: RetrieveOK=false; ProcessOK44=true;
      (default) -> OB1_N5_Wait
      STOR_Ctrl.FB5_Retrieve.OB1_N6_NEG_ProcOK -> OB1_N5_Wait : [~CRouteIn44]
      OB1_N5_Wait -> N1_T2_SPEXT : [StorInit && STOR_MODE == 2 && CRouteIn44 && KeyPos41]
      N1_T2_SPEXT -> STOR_Ctrl.FB5_Retrieve.OB1_N6_NEG_ProcOK : after(T_STOR_T2,sec)
    state OB1_N7_T3_CRouteOut [parallel]
      settings: executionOrder=4
      state OB1_N7_Wait
      state OB1_N7_Pulse
        entry: RouteOut44=true; SimASi_40.SR_44_CRoute_Out=true;
      state OB1_N7_Hold
        entry: RouteOut44=false; SimASi_40.SR_44_CRoute_Out=false;
      (default) -> OB1_N7_Wait
      OB1_N7_Hold -> OB1_N7_Wait : [~ProcessOK44]
      OB1_N7_Wait -> OB1_N7_Pulse : [KeyPos41 && ProcessOK44]
      OB1_N7_Pulse -> OB1_N7_Hold [order 1] : after(T_STOR_T3,sec)
      OB1_N7_Pulse -> OB1_N7_Hold [order 2] : [~ProcessOK44]
    state OB1_N8_N9_FB3_Map40 [parallel]
      settings: executionOrder=5
      state Map40
        en, du: SimASi_40.SR_44_No_Cart = ~CartStat28; SimASi_40.SR_44_Cart_Full = CartStat28 && Optic28; SimASi_40.SR_44_CRoute_In = CRouteIn44;
        SimActuators_40.SA_41_Led_Start = StorInit && KeyPos41; SimActuators_40.SA_41_Led_Extra1 = ~CartStat28 && KeyPos41; SimActuators_40.SA_41_Led_Extra2 = CartStat28 && Optic28 && KeyPos41;
      (default) -> Map40
  state STOR_Panel [parallel]
    entry: KeyPos41=true; SimSensors_40.SS_41_Key_Pos=true; SimSensors_40.SS_41_Start=false; SimSensors_40.SS_41_Stop=true; SimSensors_40.SS_41_Reset=false;
    SimSensors_40.SS_41_Panel_I4=false; SimSensors_40.SS_41_Panel_I5=false; SimSensors_40.SS_41_Panel_I6=false; SimSensors_40.SS_41_Panel_I7=false;
    settings: executionOrder=20
    state STOR_Rest
    (default) -> STOR_Rest
  state CONV_Plant [parallel]
    entry: ControlerOn=true; cs=6; cf=6; ct=1; tHop=0; cartPart=false;
    settings: executionOrder=1
    state Cart [parallel]
      settings: executionOrder=1
      state Cart_AtStop
      state Cart_Move
        entry: tHop = 0;
        during: if ConvOn22, tHop = tHop + Ts_SIM; end
        Cart_Move -> Cart_Move [order 1] : [tHop >= T_HOP_ARR(cf) && ((ct == 1 && PistBck24) || (ct == 2 && PistBck25) || (ct == 3 && PistBck26) || (ct == 4 && PistBck27) || (ct == 5 && PistBck28) || (ct == 6 && PistBck29))]{cf = ct; ct = mod(ct,6) + 1;}
      (default) -> Cart_AtStop
      Cart_Move -> Cart_AtStop [order 1] : [tHop >= T_HOP_ARR(cf) && ~((ct == 1 && PistBck24) || (ct == 2 && PistBck25) || (ct == 3 && PistBck26) || (ct == 4 && PistBck27) || (ct == 5 && PistBck28) || (ct == 6 && PistBck29))]{cs = ct;}
      Cart_AtStop -> Cart_Move : [ConvOn22 && ((cs == 1 && PistBck24) || (cs == 2 && PistBck25) || (cs == 3 && PistBck26) || (cs == 4 && PistBck27) || (cs == 5 && PistBck28) || (cs == 6 && PistBck29))]{cf = cs; ct = mod(cs,6) + 1; nTest = nTest + double(cs == 1 && cartPart); nProc25Done = nProc25Done + double(cs == 2 && cartPart); nRobDone = nRobDone + double(cs == 4); nStorDone = nStorDone + double(cs == 5); nLoop = nLoop + double(cs == 6); cs = 0;}
    state Pin24 [parallel]
      settings: executionOrder=3
      state Pin24_Fwd
        entry: PistBck24=false;
      state Pin24_ToBck
      state Pin24_Bck
        entry: PistBck24=true;
      state Pin24_ToFwd
      (default) -> Pin24_Fwd
      Pin24_ToFwd -> Pin24_Fwd : after(t_pin_fwd,sec)
      Pin24_Fwd -> Pin24_ToBck : [PinCmd24]
      Pin24_ToBck -> Pin24_Bck : after(t_pin_bck,sec)
      Pin24_Bck -> Pin24_ToFwd : [~PinCmd24]
    state Pin25 [parallel]
      settings: executionOrder=4
      state Pin25_Fwd
        entry: PistBck25=false;
      state Pin25_ToBck
      state Pin25_Bck
        entry: PistBck25=true;
      state Pin25_ToFwd
      (default) -> Pin25_Fwd
      Pin25_ToFwd -> Pin25_Fwd : after(t_pin_fwd,sec)
      Pin25_Fwd -> Pin25_ToBck : [PinCmd25]
      Pin25_ToBck -> Pin25_Bck : after(t_pin_bck,sec)
      Pin25_Bck -> Pin25_ToFwd : [~PinCmd25]
    state Pin26 [parallel]
      settings: executionOrder=5
      state Pin26_Fwd
        entry: PistBck26=false;
      state Pin26_ToBck
      state Pin26_Bck
        entry: PistBck26=true;
      state Pin26_ToFwd
      (default) -> Pin26_Fwd
      Pin26_ToFwd -> Pin26_Fwd : after(t_pin_fwd,sec)
      Pin26_Fwd -> Pin26_ToBck : [PinCmd26]
      Pin26_ToBck -> Pin26_Bck : after(t_pin_bck,sec)
      Pin26_Bck -> Pin26_ToFwd : [~PinCmd26]
    state Pin27 [parallel]
      settings: executionOrder=6
      state Pin27_Fwd
        entry: PistBck27=false;
      state Pin27_ToBck
      state Pin27_Bck
        entry: PistBck27=true;
      state Pin27_ToFwd
      (default) -> Pin27_Fwd
      Pin27_ToFwd -> Pin27_Fwd : after(t_pin_fwd,sec)
      Pin27_Fwd -> Pin27_ToBck : [PinCmd27]
      Pin27_ToBck -> Pin27_Bck : after(t_pin_bck,sec)
      Pin27_Bck -> Pin27_ToFwd : [~PinCmd27]
    state Stop_Sensors [parallel]
      settings: executionOrder=2
      state Sens_Map
        en, du: CartStat24 = (cs == 1) || (cs == 0 && cf == 1 && tHop < T_HOP_STATOFF(1));
        Optic24 = cartPart && ((cs == 1) || (cs == 0 && cf == 1 && tHop < T_HOP_OPTOFF(1)) || (cs == 0 && ct == 1 && tHop >= T_HOP_ARR(cf) - T_OPT_ON(1)));
        CartNext24 = (cs == 0 && cf == 1 && tHop >= T_HOP_NEXT(1) && tHop < T_HOP_NEXT(1) + T_HOP_NEXTDUR(1));
        tcnt = tHop - (T_HOP_ARR(cf) - T_CNT(1)); Count24 = (cs == 0 && ct == 1 && tcnt >= 0 && tcnt < CART_ID*t_cnt_per && mod(tcnt, t_cnt_per) < t_cnt_pulse);
        SimSensors_20.SS_24_Cart_Stat = CartStat24; SimSensors_20.SS_24_Optic = Optic24; SimSensors_20.SS_24_Cart_Next = CartNext24; SimSensors_20.SS_24_Count = Count24; SimSensors_20.SS_24_Pist_Bck = PistBck24;
        CartStat25 = (cs == 2) || (cs == 0 && cf == 2 && tHop < T_HOP_STATOFF(2));
        Optic25 = cartPart && ((cs == 2) || (cs == 0 && cf == 2 && tHop < T_HOP_OPTOFF(2)) || (cs == 0 && ct == 2 && tHop >= T_HOP_ARR(cf) - T_OPT_ON(2)));
        CartNext25 = (cs == 0 && cf == 2 && tHop >= T_HOP_NEXT(2) && tHop < T_HOP_NEXT(2) + T_HOP_NEXTDUR(2));
        tcnt = tHop - (T_HOP_ARR(cf) - T_CNT(2)); Count25 = (cs == 0 && ct == 2 && tcnt >= 0 && tcnt < CART_ID*t_cnt_per && mod(tcnt, t_cnt_per) < t_cnt_pulse);
        SimSensors_20.SS_25_Cart_Stat = CartStat25; SimSensors_20.SS_25_Optic = Optic25; SimSensors_20.SS_25_Cart_Next = CartNext25; SimSensors_20.SS_25_Count = Count25; SimSensors_20.SS_25_Pist_Bck = PistBck25;
        CartStat26 = (cs == 3) || (cs == 0 && cf == 3 && tHop < T_HOP_STATOFF(3));
        Optic26 = cartPart && ((cs == 3) || (cs == 0 && cf == 3 && tHop < T_HOP_OPTOFF(3)) || (cs == 0 && ct == 3 && tHop >= T_HOP_ARR(cf) - T_OPT_ON(3)));
        CartNext26 = (cs == 0 && cf == 3 && tHop >= T_HOP_NEXT(3) && tHop < T_HOP_NEXT(3) + T_HOP_NEXTDUR(3));
        tcnt = tHop - (T_HOP_ARR(cf) - T_CNT(3)); Count26 = (cs == 0 && ct == 3 && tcnt >= 0 && tcnt < CART_ID*t_cnt_per && mod(tcnt, t_cnt_per) < t_cnt_pulse);
        SimSensors_20.SS_26_Cart_Stat = CartStat26; SimSensors_20.SS_26_Optic = Optic26; SimSensors_20.SS_26_Cart_Next = CartNext26; SimSensors_20.SS_26_Count = Count26; SimSensors_20.SS_26_Pist_Bck = PistBck26;
        CartStat27 = (cs == 4) || (cs == 0 && cf == 4 && tHop < T_HOP_STATOFF(4));
        Optic27 = cartPart && ((cs == 4) || (cs == 0 && cf == 4 && tHop < T_HOP_OPTOFF(4)) || (cs == 0 && ct == 4 && tHop >= T_HOP_ARR(cf) - T_OPT_ON(4)));
        CartNext27 = (cs == 0 && cf == 4 && tHop >= T_HOP_NEXT(4) && tHop < T_HOP_NEXT(4) + T_HOP_NEXTDUR(4));
        tcnt = tHop - (T_HOP_ARR(cf) - T_CNT(4)); Count27 = (cs == 0 && ct == 4 && tcnt >= 0 && tcnt < CART_ID*t_cnt_per && mod(tcnt, t_cnt_per) < t_cnt_pulse);
        SimSensors_20.SS_27_Cart_Stat = CartStat27; SimSensors_20.SS_27_Optic = Optic27; SimSensors_20.SS_27_Cart_Next = CartNext27; SimSensors_20.SS_27_Count = Count27; SimSensors_20.SS_27_Pist_Bck = PistBck27;
        CartStat28 = (cs == 5) || (cs == 0 && cf == 5 && tHop < T_HOP_STATOFF(5));
        Optic28 = cartPart && ((cs == 5) || (cs == 0 && cf == 5 && tHop < T_HOP_OPTOFF(5)) || (cs == 0 && ct == 5 && tHop >= T_HOP_ARR(cf) - T_OPT_ON(5)));
        CartNext28 = (cs == 0 && cf == 5 && tHop >= T_HOP_NEXT(5) && tHop < T_HOP_NEXT(5) + T_HOP_NEXTDUR(5));
        tcnt = tHop - (T_HOP_ARR(cf) - T_CNT(5)); Count28 = (cs == 0 && ct == 5 && tcnt >= 0 && tcnt < CART_ID*t_cnt_per && mod(tcnt, t_cnt_per) < t_cnt_pulse);
        SimSensors_20.SS_28_Cart_Stat = CartStat28; SimSensors_20.SS_28_Optic = Optic28; SimSensors_20.SS_28_Cart_Next = CartNext28; SimSensors_20.SS_28_Count = Count28; SimSensors_20.SS_28_Pist_Bck = PistBck28;
        CartAt29 = (cs == 6) || (cs == 0 && cf == 6 && tHop < T_HOP_STATOFF(6));
        Optic29 = cartPart && ((cs == 6) || (cs == 0 && cf == 6 && tHop < T_HOP_OPTOFF(6)) || (cs == 0 && ct == 6 && tHop >= T_HOP_ARR(cf) - T_OPT_ON(6)));
        CartNext29 = (cs == 0 && cf == 6 && tHop >= T_HOP_NEXT(6) && tHop < T_HOP_NEXT(6) + T_HOP_NEXTDUR(6));
        tcnt = tHop - (T_HOP_ARR(cf) - T_CNT(6)); Count29 = (cs == 0 && ct == 6 && tcnt >= 0 && tcnt < CART_ID*t_cnt_per && mod(tcnt, t_cnt_per) < t_cnt_pulse);
        SimSensors_20.SS_29_Cart_Stat = CartAt29; SimSensors_20.SS_29_Optic = Optic29; SimSensors_20.SS_29_Cart_Next = CartNext29; SimSensors_20.SS_29_Count = Count29; SimSensors_20.SS_29_Pist_Bck = PistBck29;
        CartHasPart = CartStat24 && cartPart; CartHasPart25 = CartStat25 && cartPart; PartOnCart = CartAt29 && cartPart;
        SimSensors_20.SS_20_On=false; SimSensors_20.SS_20_Off=false; SimSensors_20.SS_20_Controler_On = ControlerOn;
      (default) -> CONV_Plant.Stop_Sensors.Sens_Map
    state Pin28 [parallel]
      settings: executionOrder=7
      state Pin28_Fwd
        entry: PistBck28=false;
      state Pin28_ToBck
      state Pin28_Bck
        entry: PistBck28=true;
      state Pin28_ToFwd
      (default) -> Pin28_Fwd
      Pin28_ToFwd -> Pin28_Fwd : after(t_pin_fwd,sec)
      Pin28_Fwd -> Pin28_ToBck : [PinCmd28]
      Pin28_ToBck -> Pin28_Bck : after(t_pin_bck,sec)
      Pin28_Bck -> Pin28_ToFwd : [~PinCmd28]
    state Pin29 [parallel]
      settings: executionOrder=8
      state Pin29_Fwd
        entry: PistBck29=false;
      state Pin29_ToBck
      state Pin29_Bck
        entry: PistBck29=true;
      state Pin29_ToFwd
      (default) -> Pin29_Fwd
      Pin29_ToFwd -> Pin29_Fwd : after(t_pin_fwd,sec)
      Pin29_Fwd -> Pin29_ToBck : [PinCmd29]
      Pin29_ToBck -> Pin29_Bck : after(t_pin_bck,sec)
      Pin29_Bck -> Pin29_ToFwd : [~PinCmd29]
  state FB11_Ctrl [parallel]
    entry: Selected11=false; ConvOn22=false; ConvErr22=false;
    settings: executionOrder=8
    state FB11_Dest24_Test [parallel]
      settings: executionOrder=1
      state N1_Wait
      state N1_Request
        entry: Req11_Test=true;
      state N2_PathFrom29
        entry: Path11_Test_Sort=true; Selected11=true;
      state N2_PathFrom28
        entry: Path11_Test_Stor=true; Selected11=true;
      state N2_PathFrom27
        entry: Path11_Test_Robo=true; Selected11=true;
      state N2_PathFrom26
        entry: Path11_Test_Visi=true; Selected11=true;
      state N2_PathFrom25
        entry: Path11_Test_Proc=true; Selected11=true;
      state N3_Conveyor
        entry: Conv11_Test = ControlerOn; ConvErr22 = ~ControlerOn;
      state N4_PinsOff
        entry: Path11_Test_Sort=false; Path11_Test_Stor=false; Path11_Test_Robo=false; Path11_Test_Visi=false; Path11_Test_Proc=false;
      state N6_T_SE_CartDel
        entry: Conv11_Test=false; Req11_Test=false; Selected11=false; CartDel11_Test=true;
      state N7_CartDelOff
        entry: CartDel11_Test=false;
      (default) -> FB11_Ctrl.FB11_Dest24_Test.N1_Wait
      FB11_Ctrl.FB11_Dest24_Test.N7_CartDelOff -> FB11_Ctrl.FB11_Dest24_Test.N1_Wait
      FB11_Ctrl.FB11_Dest24_Test.N1_Wait -> FB11_Ctrl.FB11_Dest24_Test.N1_Request : [ReqIn_Test && ~Req11_Proc && ~Req11_Visi && ~Req11_Robo && ~Req11_Stor && ~Req11_Sort]
      FB11_Ctrl.FB11_Dest24_Test.N1_Request -> FB11_Ctrl.FB11_Dest24_Test.N2_PathFrom29 [order 1] : [~Selected11 && CartAt29]
      FB11_Ctrl.FB11_Dest24_Test.N1_Request -> FB11_Ctrl.FB11_Dest24_Test.N2_PathFrom28 [order 2] : [~Selected11 && ~CartAt29 && CartStat28]
      FB11_Ctrl.FB11_Dest24_Test.N1_Request -> FB11_Ctrl.FB11_Dest24_Test.N2_PathFrom27 [order 3] : [~Selected11 && ~CartAt29 && ~CartStat28 && CartStat27]
      FB11_Ctrl.FB11_Dest24_Test.N1_Request -> FB11_Ctrl.FB11_Dest24_Test.N2_PathFrom26 [order 4] : [~Selected11 && ~CartAt29 && ~CartStat28 && ~CartStat27 && CartStat26]
      FB11_Ctrl.FB11_Dest24_Test.N1_Request -> FB11_Ctrl.FB11_Dest24_Test.N2_PathFrom25 [order 5] : [~Selected11 && ~CartAt29 && ~CartStat28 && ~CartStat27 && ~CartStat26]
      FB11_Ctrl.FB11_Dest24_Test.N2_PathFrom29 -> FB11_Ctrl.FB11_Dest24_Test.N3_Conveyor
      FB11_Ctrl.FB11_Dest24_Test.N2_PathFrom28 -> FB11_Ctrl.FB11_Dest24_Test.N3_Conveyor
      FB11_Ctrl.FB11_Dest24_Test.N2_PathFrom27 -> FB11_Ctrl.FB11_Dest24_Test.N3_Conveyor
      FB11_Ctrl.FB11_Dest24_Test.N2_PathFrom26 -> FB11_Ctrl.FB11_Dest24_Test.N3_Conveyor
      FB11_Ctrl.FB11_Dest24_Test.N2_PathFrom25 -> FB11_Ctrl.FB11_Dest24_Test.N3_Conveyor
      FB11_Ctrl.FB11_Dest24_Test.N3_Conveyor -> FB11_Ctrl.FB11_Dest24_Test.N4_PinsOff : [CartNext29]
      FB11_Ctrl.FB11_Dest24_Test.N4_PinsOff -> FB11_Ctrl.FB11_Dest24_Test.N6_T_SE_CartDel : [CartStat24]
      FB11_Ctrl.FB11_Dest24_Test.N6_T_SE_CartDel -> FB11_Ctrl.FB11_Dest24_Test.N7_CartDelOff : after(T_FB11_T,sec)
    state FB11_Dest25_Proc [parallel]
      settings: executionOrder=2
      state N1_Wait
      state N1_Request
        entry: Req11_Proc=true;
      state N2_PathFrom24
        entry: Path11_Proc_Test=true; Selected11=true;
      state N2_PathFrom29
        entry: Path11_Proc_Sort=true; Selected11=true;
      state N2_PathFrom28
        entry: Path11_Proc_Stor=true; Selected11=true;
      state N2_PathFrom27
        entry: Path11_Proc_Robo=true; Selected11=true;
      state N2_PathFrom26
        entry: Path11_Proc_Visi=true; Selected11=true;
      state N3_Conveyor
        entry: Conv11_Proc = ControlerOn; ConvErr22 = ~ControlerOn;
      state N4_PinsOff
        entry: Path11_Proc_Test=false; Path11_Proc_Sort=false; Path11_Proc_Stor=false; Path11_Proc_Robo=false; Path11_Proc_Visi=false;
      state N6_T_SE_CartDel
        entry: Conv11_Proc=false; Req11_Proc=false; Selected11=false; CartDel11_Proc=true;
      state N7_CartDelOff
        entry: CartDel11_Proc=false;
      (default) -> FB11_Ctrl.FB11_Dest25_Proc.N1_Wait
      FB11_Ctrl.FB11_Dest25_Proc.N7_CartDelOff -> FB11_Ctrl.FB11_Dest25_Proc.N1_Wait
      FB11_Ctrl.FB11_Dest25_Proc.N1_Wait -> FB11_Ctrl.FB11_Dest25_Proc.N1_Request : [ReqIn_Proc && ~Req11_Test && ~Req11_Visi && ~Req11_Robo && ~Req11_Stor && ~Req11_Sort]
      FB11_Ctrl.FB11_Dest25_Proc.N1_Request -> FB11_Ctrl.FB11_Dest25_Proc.N2_PathFrom24 [order 1] : [~Selected11 && CartStat24]
      FB11_Ctrl.FB11_Dest25_Proc.N1_Request -> FB11_Ctrl.FB11_Dest25_Proc.N2_PathFrom29 [order 2] : [~Selected11 && ~CartStat24 && CartAt29]
      FB11_Ctrl.FB11_Dest25_Proc.N1_Request -> FB11_Ctrl.FB11_Dest25_Proc.N2_PathFrom28 [order 3] : [~Selected11 && ~CartStat24 && ~CartAt29 && CartStat28]
      FB11_Ctrl.FB11_Dest25_Proc.N1_Request -> FB11_Ctrl.FB11_Dest25_Proc.N2_PathFrom27 [order 4] : [~Selected11 && ~CartStat24 && ~CartAt29 && ~CartStat28 && CartStat27]
      FB11_Ctrl.FB11_Dest25_Proc.N1_Request -> FB11_Ctrl.FB11_Dest25_Proc.N2_PathFrom26 [order 5] : [~Selected11 && ~CartStat24 && ~CartAt29 && ~CartStat28 && ~CartStat27]
      FB11_Ctrl.FB11_Dest25_Proc.N2_PathFrom24 -> FB11_Ctrl.FB11_Dest25_Proc.N3_Conveyor
      FB11_Ctrl.FB11_Dest25_Proc.N2_PathFrom29 -> FB11_Ctrl.FB11_Dest25_Proc.N3_Conveyor
      FB11_Ctrl.FB11_Dest25_Proc.N2_PathFrom28 -> FB11_Ctrl.FB11_Dest25_Proc.N3_Conveyor
      FB11_Ctrl.FB11_Dest25_Proc.N2_PathFrom27 -> FB11_Ctrl.FB11_Dest25_Proc.N3_Conveyor
      FB11_Ctrl.FB11_Dest25_Proc.N2_PathFrom26 -> FB11_Ctrl.FB11_Dest25_Proc.N3_Conveyor
      FB11_Ctrl.FB11_Dest25_Proc.N3_Conveyor -> FB11_Ctrl.FB11_Dest25_Proc.N4_PinsOff : [CartNext24]
      FB11_Ctrl.FB11_Dest25_Proc.N4_PinsOff -> FB11_Ctrl.FB11_Dest25_Proc.N6_T_SE_CartDel : [CartStat25]
      FB11_Ctrl.FB11_Dest25_Proc.N6_T_SE_CartDel -> FB11_Ctrl.FB11_Dest25_Proc.N7_CartDelOff : after(T_FB11_T,sec)
    state FB11_Dest26_Visi [parallel]
      settings: executionOrder=3
      state N1_Wait
      state N1_Request
        entry: Req11_Visi=true;
      state N2_PathFrom25
        entry: Path11_Visi_Proc=true; Selected11=true;
      state N2_PathFrom24
        entry: Path11_Visi_Test=true; Selected11=true;
      state N2_PathFrom29
        entry: Path11_Visi_Sort=true; Selected11=true;
      state N2_PathFrom28
        entry: Path11_Visi_Stor=true; Selected11=true;
      state N2_PathFrom27
        entry: Path11_Visi_Robo=true; Selected11=true;
      state N3_Conveyor
        entry: Conv11_Visi = ControlerOn; ConvErr22 = ~ControlerOn;
      state N4_PinsOff
        entry: Path11_Visi_Proc=false; Path11_Visi_Test=false; Path11_Visi_Sort=false; Path11_Visi_Stor=false; Path11_Visi_Robo=false;
      state N6_T_SE_CartDel
        entry: Conv11_Visi=false; Req11_Visi=false; Selected11=false; CartDel11_Visi=true;
      state N7_CartDelOff
        entry: CartDel11_Visi=false;
      (default) -> FB11_Ctrl.FB11_Dest26_Visi.N1_Wait
      FB11_Ctrl.FB11_Dest26_Visi.N7_CartDelOff -> FB11_Ctrl.FB11_Dest26_Visi.N1_Wait
      FB11_Ctrl.FB11_Dest26_Visi.N1_Wait -> FB11_Ctrl.FB11_Dest26_Visi.N1_Request : [ReqIn_Visi && ~Req11_Test && ~Req11_Proc && ~Req11_Robo && ~Req11_Stor && ~Req11_Sort]
      FB11_Ctrl.FB11_Dest26_Visi.N1_Request -> FB11_Ctrl.FB11_Dest26_Visi.N2_PathFrom25 [order 1] : [~Selected11 && CartStat25]
      FB11_Ctrl.FB11_Dest26_Visi.N1_Request -> FB11_Ctrl.FB11_Dest26_Visi.N2_PathFrom24 [order 2] : [~Selected11 && ~CartStat25 && CartStat24]
      FB11_Ctrl.FB11_Dest26_Visi.N1_Request -> FB11_Ctrl.FB11_Dest26_Visi.N2_PathFrom29 [order 3] : [~Selected11 && ~CartStat25 && ~CartStat24 && CartAt29]
      FB11_Ctrl.FB11_Dest26_Visi.N1_Request -> FB11_Ctrl.FB11_Dest26_Visi.N2_PathFrom28 [order 4] : [~Selected11 && ~CartStat25 && ~CartStat24 && ~CartAt29 && CartStat28]
      FB11_Ctrl.FB11_Dest26_Visi.N1_Request -> FB11_Ctrl.FB11_Dest26_Visi.N2_PathFrom27 [order 5] : [~Selected11 && ~CartStat25 && ~CartStat24 && ~CartAt29 && ~CartStat28]
      FB11_Ctrl.FB11_Dest26_Visi.N2_PathFrom25 -> FB11_Ctrl.FB11_Dest26_Visi.N3_Conveyor
      FB11_Ctrl.FB11_Dest26_Visi.N2_PathFrom24 -> FB11_Ctrl.FB11_Dest26_Visi.N3_Conveyor
      FB11_Ctrl.FB11_Dest26_Visi.N2_PathFrom29 -> FB11_Ctrl.FB11_Dest26_Visi.N3_Conveyor
      FB11_Ctrl.FB11_Dest26_Visi.N2_PathFrom28 -> FB11_Ctrl.FB11_Dest26_Visi.N3_Conveyor
      FB11_Ctrl.FB11_Dest26_Visi.N2_PathFrom27 -> FB11_Ctrl.FB11_Dest26_Visi.N3_Conveyor
      FB11_Ctrl.FB11_Dest26_Visi.N3_Conveyor -> FB11_Ctrl.FB11_Dest26_Visi.N4_PinsOff : [CartNext25]
      FB11_Ctrl.FB11_Dest26_Visi.N4_PinsOff -> FB11_Ctrl.FB11_Dest26_Visi.N6_T_SE_CartDel : [CartStat26]
      FB11_Ctrl.FB11_Dest26_Visi.N6_T_SE_CartDel -> FB11_Ctrl.FB11_Dest26_Visi.N7_CartDelOff : after(T_FB11_T,sec)
    state FB11_Dest27_Robo [parallel]
      settings: executionOrder=4
      state N1_Wait
      state N1_Request
        entry: Req11_Robo=true;
      state N2_PathFrom26
        entry: Path11_Robo_Visi=true; Selected11=true;
      state N2_PathFrom25
        entry: Path11_Robo_Proc=true; Selected11=true;
      state N2_PathFrom24
        entry: Path11_Robo_Test=true; Selected11=true;
      state N2_PathFrom29
        entry: Path11_Robo_Sort=true; Selected11=true;
      state N2_PathFrom28
        entry: Path11_Robo_Stor=true; Selected11=true;
      state N3_Conveyor
        entry: Conv11_Robo = ControlerOn; ConvErr22 = ~ControlerOn;
      state N4_PinsOff
        entry: Path11_Robo_Visi=false; Path11_Robo_Proc=false; Path11_Robo_Test=false; Path11_Robo_Sort=false; Path11_Robo_Stor=false;
      state N6_T_SE_CartDel
        entry: Conv11_Robo=false; Req11_Robo=false; Selected11=false; CartDel11_Robo=true;
      state N7_CartDelOff
        entry: CartDel11_Robo=false;
      (default) -> FB11_Ctrl.FB11_Dest27_Robo.N1_Wait
      FB11_Ctrl.FB11_Dest27_Robo.N7_CartDelOff -> FB11_Ctrl.FB11_Dest27_Robo.N1_Wait
      FB11_Ctrl.FB11_Dest27_Robo.N1_Wait -> FB11_Ctrl.FB11_Dest27_Robo.N1_Request : [ReqIn_Robo && ~Req11_Test && ~Req11_Proc && ~Req11_Visi && ~Req11_Stor && ~Req11_Sort]
      FB11_Ctrl.FB11_Dest27_Robo.N1_Request -> FB11_Ctrl.FB11_Dest27_Robo.N2_PathFrom26 [order 1] : [~Selected11 && CartStat26]
      FB11_Ctrl.FB11_Dest27_Robo.N1_Request -> FB11_Ctrl.FB11_Dest27_Robo.N2_PathFrom25 [order 2] : [~Selected11 && ~CartStat26 && CartStat25]
      FB11_Ctrl.FB11_Dest27_Robo.N1_Request -> FB11_Ctrl.FB11_Dest27_Robo.N2_PathFrom24 [order 3] : [~Selected11 && ~CartStat26 && ~CartStat25 && CartStat24]
      FB11_Ctrl.FB11_Dest27_Robo.N1_Request -> FB11_Ctrl.FB11_Dest27_Robo.N2_PathFrom29 [order 4] : [~Selected11 && ~CartStat26 && ~CartStat25 && ~CartStat24 && CartAt29]
      FB11_Ctrl.FB11_Dest27_Robo.N1_Request -> FB11_Ctrl.FB11_Dest27_Robo.N2_PathFrom28 [order 5] : [~Selected11 && ~CartStat26 && ~CartStat25 && ~CartStat24 && ~CartAt29]
      FB11_Ctrl.FB11_Dest27_Robo.N2_PathFrom26 -> FB11_Ctrl.FB11_Dest27_Robo.N3_Conveyor
      FB11_Ctrl.FB11_Dest27_Robo.N2_PathFrom25 -> FB11_Ctrl.FB11_Dest27_Robo.N3_Conveyor
      FB11_Ctrl.FB11_Dest27_Robo.N2_PathFrom24 -> FB11_Ctrl.FB11_Dest27_Robo.N3_Conveyor
      FB11_Ctrl.FB11_Dest27_Robo.N2_PathFrom29 -> FB11_Ctrl.FB11_Dest27_Robo.N3_Conveyor
      FB11_Ctrl.FB11_Dest27_Robo.N2_PathFrom28 -> FB11_Ctrl.FB11_Dest27_Robo.N3_Conveyor
      FB11_Ctrl.FB11_Dest27_Robo.N3_Conveyor -> FB11_Ctrl.FB11_Dest27_Robo.N4_PinsOff : [CartNext26]
      FB11_Ctrl.FB11_Dest27_Robo.N4_PinsOff -> FB11_Ctrl.FB11_Dest27_Robo.N6_T_SE_CartDel : [CartStat27]
      FB11_Ctrl.FB11_Dest27_Robo.N6_T_SE_CartDel -> FB11_Ctrl.FB11_Dest27_Robo.N7_CartDelOff : after(T_FB11_T,sec)
    state FB11_Dest28_Stor [parallel]
      settings: executionOrder=5
      state N1_Wait
      state N1_Request
        entry: Req11_Stor=true;
      state N2_PathFrom27
        entry: Path11_Stor_Robo=true; Selected11=true;
      state N2_PathFrom26
        entry: Path11_Stor_Visi=true; Selected11=true;
      state N2_PathFrom25
        entry: Path11_Stor_Proc=true; Selected11=true;
      state N2_PathFrom24
        entry: Path11_Stor_Test=true; Selected11=true;
      state N2_PathFrom29
        entry: Path11_Stor_Sort=true; Selected11=true;
      state N3_Conveyor
        entry: Conv11_Stor = ControlerOn; ConvErr22 = ~ControlerOn;
      state N4_PinsOff
        entry: Path11_Stor_Robo=false; Path11_Stor_Visi=false; Path11_Stor_Proc=false; Path11_Stor_Test=false; Path11_Stor_Sort=false;
      state N6_T_SE_CartDel
        entry: Conv11_Stor=false; Req11_Stor=false; Selected11=false; CartDel11_Stor=true;
      state N7_CartDelOff
        entry: CartDel11_Stor=false;
      (default) -> FB11_Ctrl.FB11_Dest28_Stor.N1_Wait
      FB11_Ctrl.FB11_Dest28_Stor.N7_CartDelOff -> FB11_Ctrl.FB11_Dest28_Stor.N1_Wait
      FB11_Ctrl.FB11_Dest28_Stor.N1_Wait -> FB11_Ctrl.FB11_Dest28_Stor.N1_Request : [ReqIn_Stor && ~Req11_Test && ~Req11_Proc && ~Req11_Visi && ~Req11_Robo && ~Req11_Sort]
      FB11_Ctrl.FB11_Dest28_Stor.N1_Request -> FB11_Ctrl.FB11_Dest28_Stor.N2_PathFrom27 [order 1] : [~Selected11 && CartStat27]
      FB11_Ctrl.FB11_Dest28_Stor.N1_Request -> FB11_Ctrl.FB11_Dest28_Stor.N2_PathFrom26 [order 2] : [~Selected11 && ~CartStat27 && CartStat26]
      FB11_Ctrl.FB11_Dest28_Stor.N1_Request -> FB11_Ctrl.FB11_Dest28_Stor.N2_PathFrom25 [order 3] : [~Selected11 && ~CartStat27 && ~CartStat26 && CartStat25]
      FB11_Ctrl.FB11_Dest28_Stor.N1_Request -> FB11_Ctrl.FB11_Dest28_Stor.N2_PathFrom24 [order 4] : [~Selected11 && ~CartStat27 && ~CartStat26 && ~CartStat25 && CartStat24]
      FB11_Ctrl.FB11_Dest28_Stor.N1_Request -> FB11_Ctrl.FB11_Dest28_Stor.N2_PathFrom29 [order 5] : [~Selected11 && ~CartStat27 && ~CartStat26 && ~CartStat25 && ~CartStat24]
      FB11_Ctrl.FB11_Dest28_Stor.N2_PathFrom27 -> FB11_Ctrl.FB11_Dest28_Stor.N3_Conveyor
      FB11_Ctrl.FB11_Dest28_Stor.N2_PathFrom26 -> FB11_Ctrl.FB11_Dest28_Stor.N3_Conveyor
      FB11_Ctrl.FB11_Dest28_Stor.N2_PathFrom25 -> FB11_Ctrl.FB11_Dest28_Stor.N3_Conveyor
      FB11_Ctrl.FB11_Dest28_Stor.N2_PathFrom24 -> FB11_Ctrl.FB11_Dest28_Stor.N3_Conveyor
      FB11_Ctrl.FB11_Dest28_Stor.N2_PathFrom29 -> FB11_Ctrl.FB11_Dest28_Stor.N3_Conveyor
      FB11_Ctrl.FB11_Dest28_Stor.N3_Conveyor -> FB11_Ctrl.FB11_Dest28_Stor.N4_PinsOff : [CartNext27]
      FB11_Ctrl.FB11_Dest28_Stor.N4_PinsOff -> FB11_Ctrl.FB11_Dest28_Stor.N6_T_SE_CartDel : [CartStat28]
      FB11_Ctrl.FB11_Dest28_Stor.N6_T_SE_CartDel -> FB11_Ctrl.FB11_Dest28_Stor.N7_CartDelOff : after(T_FB11_T,sec)
    state FB11_Dest29_Sort [parallel]
      settings: executionOrder=6
      state N1_Wait
      state N1_Request
        entry: Req11_Sort=true;
      state N2_PathFrom28
        entry: Path11_Sort_Stor=true; Selected11=true;
      state N2_PathFrom27
        entry: Path11_Sort_Robo=true; Selected11=true;
      state N2_PathFrom26
        entry: Path11_Sort_Visi=true; Selected11=true;
      state N2_PathFrom25
        entry: Path11_Sort_Proc=true; Selected11=true;
      state N2_PathFrom24
        entry: Path11_Sort_Test=true; Selected11=true;
      state N3_Conveyor
        entry: Conv11_Sort = ControlerOn; ConvErr22 = ~ControlerOn;
      state N4_PinsOff
        entry: Path11_Sort_Stor=false; Path11_Sort_Robo=false; Path11_Sort_Visi=false; Path11_Sort_Proc=false; Path11_Sort_Test=false;
      state N6_T_SE_CartDel
        entry: Conv11_Sort=false; Req11_Sort=false; Selected11=false; CartDel11_Sort=true;
      state N7_CartDelOff
        entry: CartDel11_Sort=false;
      (default) -> FB11_Ctrl.FB11_Dest29_Sort.N1_Wait
      FB11_Ctrl.FB11_Dest29_Sort.N7_CartDelOff -> FB11_Ctrl.FB11_Dest29_Sort.N1_Wait
      FB11_Ctrl.FB11_Dest29_Sort.N1_Wait -> FB11_Ctrl.FB11_Dest29_Sort.N1_Request : [ReqIn_Sort && ~Req11_Test && ~Req11_Proc && ~Req11_Visi && ~Req11_Robo && ~Req11_Stor]
      FB11_Ctrl.FB11_Dest29_Sort.N1_Request -> FB11_Ctrl.FB11_Dest29_Sort.N2_PathFrom28 [order 1] : [~Selected11 && CartStat28]
      FB11_Ctrl.FB11_Dest29_Sort.N1_Request -> FB11_Ctrl.FB11_Dest29_Sort.N2_PathFrom27 [order 2] : [~Selected11 && ~CartStat28 && CartStat27]
      FB11_Ctrl.FB11_Dest29_Sort.N1_Request -> FB11_Ctrl.FB11_Dest29_Sort.N2_PathFrom26 [order 3] : [~Selected11 && ~CartStat28 && ~CartStat27 && CartStat26]
      FB11_Ctrl.FB11_Dest29_Sort.N1_Request -> FB11_Ctrl.FB11_Dest29_Sort.N2_PathFrom25 [order 4] : [~Selected11 && ~CartStat28 && ~CartStat27 && ~CartStat26 && CartStat25]
      FB11_Ctrl.FB11_Dest29_Sort.N1_Request -> FB11_Ctrl.FB11_Dest29_Sort.N2_PathFrom24 [order 5] : [~Selected11 && ~CartStat28 && ~CartStat27 && ~CartStat26 && ~CartStat25]
      FB11_Ctrl.FB11_Dest29_Sort.N2_PathFrom28 -> FB11_Ctrl.FB11_Dest29_Sort.N3_Conveyor
      FB11_Ctrl.FB11_Dest29_Sort.N2_PathFrom27 -> FB11_Ctrl.FB11_Dest29_Sort.N3_Conveyor
      FB11_Ctrl.FB11_Dest29_Sort.N2_PathFrom26 -> FB11_Ctrl.FB11_Dest29_Sort.N3_Conveyor
      FB11_Ctrl.FB11_Dest29_Sort.N2_PathFrom25 -> FB11_Ctrl.FB11_Dest29_Sort.N3_Conveyor
      FB11_Ctrl.FB11_Dest29_Sort.N2_PathFrom24 -> FB11_Ctrl.FB11_Dest29_Sort.N3_Conveyor
      FB11_Ctrl.FB11_Dest29_Sort.N3_Conveyor -> FB11_Ctrl.FB11_Dest29_Sort.N4_PinsOff : [CartNext28]
      FB11_Ctrl.FB11_Dest29_Sort.N4_PinsOff -> FB11_Ctrl.FB11_Dest29_Sort.N6_T_SE_CartDel : [CartAt29]
      FB11_Ctrl.FB11_Dest29_Sort.N6_T_SE_CartDel -> FB11_Ctrl.FB11_Dest29_Sort.N7_CartDelOff : after(T_FB11_T,sec)
    state N5_CartID [parallel]
      settings: executionOrder=7
      state N5_Count
        en, du: if Count24 && ~CTp24, CID24 = CID24 + 1; end; if PistBck24 && ~PBp24, CID24 = 0; end; CTp24 = Count24; PBp24 = PistBck24; SimASi_70.SR_73_TestCartID = CID24;
        if Count25 && ~CTp25, CID25 = CID25 + 1; end; if PistBck25 && ~PBp25, CID25 = 0; end; CTp25 = Count25; PBp25 = PistBck25; SimASi_90.SR_93_ProcCartID = CID25;
        if Count26 && ~CTp26, CID26 = CID26 + 1; end; if PistBck26 && ~PBp26, CID26 = 0; end; CTp26 = Count26; PBp26 = PistBck26;
        if Count27 && ~CTp27, CID27 = CID27 + 1; end; if PistBck27 && ~PBp27, CID27 = 0; end; CTp27 = Count27; PBp27 = PistBck27; SimASi_30.SR_32_RoboCartID = CID27;
        if Count28 && ~CTp28, CID28 = CID28 + 1; end; if PistBck28 && ~PBp28, CID28 = 0; end; CTp28 = Count28; PBp28 = PistBck28; SimASi_40.SR_43_StorCartID = CID28;
        if Count29 && ~CTp29, CID29 = CID29 + 1; end; if PistBck29 && ~PBp29, CID29 = 0; end; CTp29 = Count29; PBp29 = PistBck29; SimASi_50.SR_53_SortCartID = CID29;
      (default) -> N5_Count
    state N43_N48_Pins_FB2 [parallel]
      settings: executionOrder=8
      state Pins_FB2_Map
        en, du: PinCmd24 = Path11_Proc_Test || Path11_Proc_Visi || Path11_Proc_Robo || Path11_Proc_Stor || Path11_Proc_Sort || Path11_Visi_Test || Path11_Visi_Robo || Path11_Visi_Stor || Path11_Visi_Sort || Path11_Robo_Test || Path11_Robo_Stor || Path11_Robo_Sort || Path11_Stor_Test || Path11_Stor_Sort || Path11_Sort_Test;
        PinCmd25 = Path11_Test_Proc || Path11_Visi_Test || Path11_Visi_Proc || Path11_Visi_Robo || Path11_Visi_Stor || Path11_Visi_Sort || Path11_Robo_Test || Path11_Robo_Proc || Path11_Robo_Stor || Path11_Robo_Sort || Path11_Stor_Test || Path11_Stor_Proc || Path11_Stor_Sort || Path11_Sort_Test || Path11_Sort_Proc;
        PinCmd26 = Path11_Test_Proc || Path11_Test_Visi || Path11_Proc_Visi || Path11_Robo_Test || Path11_Robo_Proc || Path11_Robo_Visi || Path11_Robo_Stor || Path11_Robo_Sort || Path11_Stor_Test || Path11_Stor_Proc || Path11_Stor_Visi || Path11_Stor_Sort || Path11_Sort_Test || Path11_Sort_Proc || Path11_Sort_Visi;
        PinCmd27 = Path11_Test_Proc || Path11_Test_Visi || Path11_Test_Robo || Path11_Proc_Visi || Path11_Proc_Robo || Path11_Visi_Robo || Path11_Stor_Test || Path11_Stor_Proc || Path11_Stor_Visi || Path11_Stor_Robo || Path11_Stor_Sort || Path11_Sort_Test || Path11_Sort_Proc || Path11_Sort_Visi || Path11_Sort_Robo;
        PinCmd28 = Path11_Test_Proc || Path11_Test_Visi || Path11_Test_Robo || Path11_Test_Stor || Path11_Proc_Visi || Path11_Proc_Robo || Path11_Proc_Stor || Path11_Visi_Robo || Path11_Visi_Stor || Path11_Robo_Stor || Path11_Sort_Test || Path11_Sort_Proc || Path11_Sort_Visi || Path11_Sort_Robo || Path11_Sort_Stor;
        PinCmd29 = Path11_Test_Proc || Path11_Test_Visi || Path11_Test_Robo || Path11_Test_Stor || Path11_Test_Sort || Path11_Proc_Visi || Path11_Proc_Robo || Path11_Proc_Stor || Path11_Proc_Sort || Path11_Visi_Robo || Path11_Visi_Stor || Path11_Visi_Sort || Path11_Robo_Stor || Path11_Robo_Sort || Path11_Stor_Sort;
        ConvOn22 = (Conv11_Test || Conv11_Proc || Conv11_Visi || Conv11_Robo || Conv11_Stor || Conv11_Sort) && ControlerOn;
        SimActuators_20.SA_20_Conveyor = ConvOn22; SimActuators_20.SA_20_Led_On = ControlerOn; SimActuators_20.SA_20_Led_Off = ~ControlerOn;
        SimActuators_20.SA_24_Cart_Test = PinCmd24; SimActuators_20.SA_25_Cart_Proc = PinCmd25; SimActuators_20.SA_26_Cart_Visi = PinCmd26; SimActuators_20.SA_27_Cart_Robo = PinCmd27; SimActuators_20.SA_28_Cart_Stor = PinCmd28; SimActuators_20.SA_29_Cart_Sort = PinCmd29;
        SimControl_20.SC_24_CartDel = CartDel11_Test; SimControl_20.SC_24_CRoute_Out = RouteOut74; SimControl_20.SC_25_CartDel = CartDel11_Proc; SimControl_20.SC_25_CRoute_Out = RouteOut94;
        SimControl_20.SC_26_CartDel = CartDel11_Visi; SimControl_20.SC_26_CRoute_Out = VisDone26; SimControl_20.SC_27_CartDel = CartDel11_Robo; SimControl_20.SC_27_CRoute_Out = RouteOut34;
        SimControl_20.SC_28_CartDel = CartDel11_Stor; SimControl_20.SC_28_CRoute_Out = RouteOut44; SimControl_20.SC_29_CartDel = CartDel11_Sort; SimControl_20.SC_29_CRoute_Out = RouteOut54;
      (default) -> Pins_FB2_Map
  state MES_Super [parallel]
    settings: executionOrder=16
    state MES_Start [parallel]
      settings: executionOrder=1
      state Start_Wait
      state Start_Go
        entry: MesStart=true;
      state Start_Done
        entry: MesStart=false;
      (default) -> Start_Wait
      Start_Wait -> Start_Go : after(t_mes_start,sec)
      Start_Go -> Start_Done : [ReqIn_Test]
    state MES_Req24 [parallel]
      settings: executionOrder=2
      state Req_Wait
      state Req_Delay
      state Req_Write
        entry: SimControl_20.SC_24_Request=true;
      state Req_Seen
        entry: ReqIn_Test=true;
      state Req_End
        entry: SimControl_20.SC_24_Request=false; ReqIn_Test=false;
      (default) -> MES_Super.MES_Req24.Req_Wait
      MES_Super.MES_Req24.Req_End -> MES_Super.MES_Req24.Req_Wait : [~(RouteOut54)]
      MES_Super.MES_Req24.Req_Wait -> MES_Super.MES_Req24.Req_Delay : [(RouteOut54 || MesStart) && nTest < N_PARTS]
      MES_Super.MES_Req24.Req_Delay -> MES_Super.MES_Req24.Req_Write : after(t_mes_req,sec)
      MES_Super.MES_Req24.Req_Write -> MES_Super.MES_Req24.Req_Seen : after(t_opc,sec)
      MES_Super.MES_Req24.Req_Seen -> MES_Super.MES_Req24.Req_End : after(t_mes_reqdur - t_opc,sec)
    state MES_Req25 [parallel]
      settings: executionOrder=3
      state Req_Wait
      state Req_Delay
      state Req_Write
        entry: SimControl_20.SC_25_Request=true;
      state Req_Seen
        entry: ReqIn_Proc=true;
      state Req_End
        entry: SimControl_20.SC_25_Request=false; ReqIn_Proc=false;
      (default) -> MES_Super.MES_Req25.Req_Wait
      MES_Super.MES_Req25.Req_End -> MES_Super.MES_Req25.Req_Wait : [~(RouteOut74)]
      MES_Super.MES_Req25.Req_Wait -> MES_Super.MES_Req25.Req_Delay : [RouteOut74]
      MES_Super.MES_Req25.Req_Delay -> MES_Super.MES_Req25.Req_Write : after(t_mes_req,sec)
      MES_Super.MES_Req25.Req_Write -> MES_Super.MES_Req25.Req_Seen : after(t_opc,sec)
      MES_Super.MES_Req25.Req_Seen -> MES_Super.MES_Req25.Req_End : after(t_mes_reqdur - t_opc,sec)
    state MES_Req26 [parallel]
      settings: executionOrder=4
      state Req_Wait
      state Req_Delay
      state Req_Write
        entry: SimControl_20.SC_26_Request=true;
      state Req_Seen
        entry: ReqIn_Visi=true;
      state Req_End
        entry: SimControl_20.SC_26_Request=false; ReqIn_Visi=false;
      (default) -> MES_Super.MES_Req26.Req_Wait
      MES_Super.MES_Req26.Req_End -> MES_Super.MES_Req26.Req_Wait : [~(RouteOut94)]
      MES_Super.MES_Req26.Req_Wait -> MES_Super.MES_Req26.Req_Delay : [RouteOut94]
      MES_Super.MES_Req26.Req_Delay -> MES_Super.MES_Req26.Req_Write : after(t_mes_req,sec)
      MES_Super.MES_Req26.Req_Write -> MES_Super.MES_Req26.Req_Seen : after(t_opc,sec)
      MES_Super.MES_Req26.Req_Seen -> MES_Super.MES_Req26.Req_End : after(t_mes_reqdur - t_opc,sec)
    state MES_Req27 [parallel]
      settings: executionOrder=5
      state Req_Wait
      state Req_Delay
      state Req_Write
        entry: SimControl_20.SC_27_Request=true;
      state Req_Seen
        entry: ReqIn_Robo=true;
      state Req_End
        entry: SimControl_20.SC_27_Request=false; ReqIn_Robo=false;
      (default) -> MES_Super.MES_Req27.Req_Wait
      MES_Super.MES_Req27.Req_End -> MES_Super.MES_Req27.Req_Wait : [~(VisDone26)]
      MES_Super.MES_Req27.Req_Wait -> MES_Super.MES_Req27.Req_Delay : [VisDone26]
      MES_Super.MES_Req27.Req_Delay -> MES_Super.MES_Req27.Req_Write : after(t_mes_req,sec)
      MES_Super.MES_Req27.Req_Write -> MES_Super.MES_Req27.Req_Seen : after(t_opc,sec)
      MES_Super.MES_Req27.Req_Seen -> MES_Super.MES_Req27.Req_End : after(t_mes_reqdur - t_opc,sec)
    state MES_Req28 [parallel]
      settings: executionOrder=6
      state Req_Wait
      state Req_Delay
      state Req_Write
        entry: SimControl_20.SC_28_Request=true;
      state Req_Seen
        entry: ReqIn_Stor=true;
      state Req_End
        entry: SimControl_20.SC_28_Request=false; ReqIn_Stor=false;
      (default) -> MES_Super.MES_Req28.Req_Wait
      MES_Super.MES_Req28.Req_End -> MES_Super.MES_Req28.Req_Wait : [~(RouteOut34)]
      MES_Super.MES_Req28.Req_Wait -> MES_Super.MES_Req28.Req_Delay : [RouteOut34]
      MES_Super.MES_Req28.Req_Delay -> MES_Super.MES_Req28.Req_Write : after(t_mes_req,sec)
      MES_Super.MES_Req28.Req_Write -> MES_Super.MES_Req28.Req_Seen : after(t_opc,sec)
      MES_Super.MES_Req28.Req_Seen -> MES_Super.MES_Req28.Req_End : after(t_mes_reqdur - t_opc,sec)
    state MES_Req29 [parallel]
      settings: executionOrder=7
      state Req_Wait
      state Req_Delay
      state Req_Write
        entry: SimControl_20.SC_29_Request=true;
      state Req_Seen
        entry: ReqIn_Sort=true;
      state Req_End
        entry: SimControl_20.SC_29_Request=false; ReqIn_Sort=false;
      (default) -> MES_Super.MES_Req29.Req_Wait
      MES_Super.MES_Req29.Req_End -> MES_Super.MES_Req29.Req_Wait : [~(RouteOut44)]
      MES_Super.MES_Req29.Req_Wait -> MES_Super.MES_Req29.Req_Delay : [RouteOut44]
      MES_Super.MES_Req29.Req_Delay -> MES_Super.MES_Req29.Req_Write : after(t_mes_req,sec)
      MES_Super.MES_Req29.Req_Write -> MES_Super.MES_Req29.Req_Seen : after(t_opc,sec)
      MES_Super.MES_Req29.Req_Seen -> MES_Super.MES_Req29.Req_End : after(t_mes_reqdur - t_opc,sec)
    state MES_Arr24 [parallel]
      settings: executionOrder=8
      state Arr_Wait
      state Arr_Delay
        entry: RQ1_70 = RQ_DELIVERY(min(nTest + 1, size(RQ_DELIVERY,1)), 1) == 1; RQ2_70 = RQ_DELIVERY(min(nTest + 1, size(RQ_DELIVERY,1)), 2) == 1;
        SimControl_70.SC_75_RQ_Delivery1 = RQ1_70; SimControl_70.SC_75_RQ_Delivery2 = RQ2_70;
      state Arr_CRouteIn
        entry: SimControl_20.SC_24_CRoute_In=true; CRouteIn74=true; SimASi_70.SR_74_CRoute_In=true;
      state Arr_Docked
        entry: SimControl_20.SC_24_CRoute_In=false; CRouteIn74=false; SimASi_70.SR_74_CRoute_In=false;
      (default) -> MES_Super.MES_Arr24.Arr_Wait
      MES_Super.MES_Arr24.Arr_Docked -> MES_Super.MES_Arr24.Arr_Wait : [~CartDel11_Test]
      MES_Super.MES_Arr24.Arr_Wait -> MES_Super.MES_Arr24.Arr_Delay : [CartDel11_Test]
      MES_Super.MES_Arr24.Arr_Delay -> MES_Super.MES_Arr24.Arr_CRouteIn : after(t_mes_cri0,sec)
      MES_Super.MES_Arr24.Arr_CRouteIn -> MES_Super.MES_Arr24.Arr_Docked : after(t_mes_cri,sec)
    state MES_Arr25 [parallel]
      settings: executionOrder=9
      state Arr_Wait
      state Arr_Delay
      state Arr_CRouteIn
        entry: SimControl_20.SC_25_CRoute_In=true; CRouteIn94=true;
      state Arr_Docked
        entry: SimControl_20.SC_25_CRoute_In=false; CRouteIn94=false;
      (default) -> MES_Super.MES_Arr25.Arr_Wait
      MES_Super.MES_Arr25.Arr_Docked -> MES_Super.MES_Arr25.Arr_Wait : [~CartDel11_Proc]
      MES_Super.MES_Arr25.Arr_Wait -> MES_Super.MES_Arr25.Arr_Delay : [CartDel11_Proc]
      MES_Super.MES_Arr25.Arr_Delay -> MES_Super.MES_Arr25.Arr_CRouteIn : after(t_mes_cri0,sec)
      MES_Super.MES_Arr25.Arr_CRouteIn -> MES_Super.MES_Arr25.Arr_Docked : after(t_mes_cri,sec)
    state MES_Arr26 [parallel]
      settings: executionOrder=10
      state Arr_Wait
      state Arr_Delay
      state Arr_CRouteIn
        entry: SimControl_20.SC_26_CRoute_In=true; CRouteIn26=true;
      state Arr_Docked
        entry: SimControl_20.SC_26_CRoute_In=false; CRouteIn26=false;
      (default) -> MES_Super.MES_Arr26.Arr_Wait
      MES_Super.MES_Arr26.Arr_Docked -> MES_Super.MES_Arr26.Arr_Wait : [~CartDel11_Visi]
      MES_Super.MES_Arr26.Arr_Wait -> MES_Super.MES_Arr26.Arr_Delay : [CartDel11_Visi]
      MES_Super.MES_Arr26.Arr_Delay -> MES_Super.MES_Arr26.Arr_CRouteIn : after(t_mes_cri0,sec)
      MES_Super.MES_Arr26.Arr_CRouteIn -> MES_Super.MES_Arr26.Arr_Docked : after(t_mes_cri,sec)
    state MES_Arr27 [parallel]
      settings: executionOrder=11
      state Arr_Wait
      state Arr_Delay
      state Arr_CRouteIn
        entry: SimControl_20.SC_27_CRoute_In=true; CRouteIn34=true;
      state Arr_Docked
        entry: SimControl_20.SC_27_CRoute_In=false; CRouteIn34=false;
      (default) -> MES_Super.MES_Arr27.Arr_Wait
      MES_Super.MES_Arr27.Arr_Docked -> MES_Super.MES_Arr27.Arr_Wait : [~CartDel11_Robo]
      MES_Super.MES_Arr27.Arr_Wait -> MES_Super.MES_Arr27.Arr_Delay : [CartDel11_Robo]
      MES_Super.MES_Arr27.Arr_Delay -> MES_Super.MES_Arr27.Arr_CRouteIn : after(t_mes_cri0,sec)
      MES_Super.MES_Arr27.Arr_CRouteIn -> MES_Super.MES_Arr27.Arr_Docked : after(t_mes_cri,sec)
    state MES_Arr28 [parallel]
      settings: executionOrder=12
      state Arr_Wait
      state Arr_Delay
      state Arr_CRouteIn
        entry: SimControl_20.SC_28_CRoute_In=true; CRouteIn44=true;
      state Arr_Docked
        entry: SimControl_20.SC_28_CRoute_In=false; CRouteIn44=false;
      (default) -> MES_Super.MES_Arr28.Arr_Wait
      MES_Super.MES_Arr28.Arr_Docked -> MES_Super.MES_Arr28.Arr_Wait : [~CartDel11_Stor]
      MES_Super.MES_Arr28.Arr_Wait -> MES_Super.MES_Arr28.Arr_Delay : [CartDel11_Stor]
      MES_Super.MES_Arr28.Arr_Delay -> MES_Super.MES_Arr28.Arr_CRouteIn : after(t_mes_cri0,sec)
      MES_Super.MES_Arr28.Arr_CRouteIn -> MES_Super.MES_Arr28.Arr_Docked : after(t_mes_cri,sec)
    state MES_Arr29 [parallel]
      settings: executionOrder=13
      state Arr_Wait
      state Arr_Delay
      state Arr_CRouteIn
        entry: SimControl_20.SC_29_CRoute_In=true; CRouteIn54=true; SimASi_50.SR_54_CRoute_In=true;
      state Arr_Docked
        entry: SimControl_20.SC_29_CRoute_In=false; CRouteIn54=false; SimASi_50.SR_54_CRoute_In=false;
      (default) -> MES_Super.MES_Arr29.Arr_Wait
      MES_Super.MES_Arr29.Arr_Docked -> MES_Super.MES_Arr29.Arr_Wait : [~CartDel11_Sort]
      MES_Super.MES_Arr29.Arr_Wait -> MES_Super.MES_Arr29.Arr_Delay : [CartDel11_Sort]
      MES_Super.MES_Arr29.Arr_Delay -> MES_Super.MES_Arr29.Arr_CRouteIn : after(t_mes_cri0,sec)
      MES_Super.MES_Arr29.Arr_CRouteIn -> MES_Super.MES_Arr29.Arr_Docked : after(t_mes_cri,sec)
  state VISION_Stn [parallel]
    settings: executionOrder=19
    state Vis_Wait
      entry: VisDone26=false;
    state Vis_Inspect
    state Vis_Done
      entry: VisDone26=true;
    (default) -> Vis_Wait
    Vis_Done -> Vis_Wait : [~CartStat26]
    Vis_Wait -> Vis_Inspect : [CartStat26]
    Vis_Inspect -> Vis_Done : after(t_vis - t_mes_req,sec)
  data: SimActuators_20 output Bus: B_SimActuators_20; SimControl_20 output Bus: B_SimControl_20; SimSensors_20 output Bus: B_SimSensors_20; SimActuators_50 output Bus: B_SimActuators_50; SimASi_50 output Bus: B_SimASi_50; SimControl_50 output Bus: B_SimControl_50; SimSensors_50 output Bus: B_SimSensors_50; SimActuators_60 output Bus: B_SimActuators_60; SimControl_60 output Bus: B_SimControl_60; SimSensors_60 output Bus: B_SimSensors_60; Ts_SIM parameter double; T_HD1_T1 parameter double; T_CONV_T6 parameter double; t_v_down parameter double; t_v_up parameter double; t_h_del parameter double; t_h_cart parameter double; t_grip parameter double; t_conv parameter double; t_leave parameter double; N_PARTS parameter double; SORT_MODE parameter double; T_SORT_ID parameter double; T_SORT_T7 parameter double; t_s_spart_off parameter double; t_s_photo parameter double; t_s_ind parameter double; t_s_ind_off parameter double; t_s_photo_off parameter double; t_s_pass1 parameter double; t_s_pass2 parameter double; t_s_pass3 parameter double; t_s_pp parameter double; t_sl1_fwd parameter double; t_sl1_bck parameter double; t_sl2_fwd parameter double; t_sl2_bck parameter double; PART_COLORS parameter double; SORT_MAP parameter double; PartOnCart local boolean =false; CartAt29 local boolean =false; CRouteIn54 local boolean =false; Claw2CartCmd local boolean =false; FB1Init local boolean =false; FB1Conv local boolean =false; FB1IDPin local boolean =false; FBSel local boolean =false; ConvOn60 local boolean =false; TrigConv local boolean =false; Lever1 local boolean =false; Lever2 local boolean =false; PassStr local boolean =false; PinSort local boolean =false; PartDel local boolean =false; nCart local double =0; nDone local double =0; nSortIn local double =0; sortColor local double =0; sortExit local double =0; cID local double =0; xSort local double =0; SimActuators_70 output Bus: B_SimActuators_70; SimASi_70 output Bus: B_SimASi_70; SimControl_70 output Bus: B_SimControl_70; SimSensors_70 output Bus: B_SimSensors_70; TEST_MODE parameter double; T_TEST_T1 parameter double; T_TEST_T2 parameter double; T_TEST_T8 parameter double; T_TEST_T3 parameter double; T_TEST_T5 parameter double; T_TEST_T6 parameter double; T_TEST_T7 parameter double; T_CONV24_T1 parameter double; t_t_up parameter double; t_t_up_lowoff parameter double; t_t_up_ind parameter double; t_t_up_sst parameter double; t_t_metal_off parameter double; t_t_height_pre parameter double; t_t_down parameter double; t_t_down_highoff parameter double; t_t_down_sst parameter double; t_t_down_ind parameter double; t_t_ej_spart parameter double; t_t_pist_fwd parameter double; t_t_pist_back parameter double; t_t_ej_cart parameter double; t_24_arrive parameter double; t_24_count parameter double; t_24_req parameter double; t_24_croute_in0 parameter double; t_24_croute_in parameter double; t_24_pist_bck parameter double; t_24_optic_off parameter double; t_24_leave parameter double; RQ_DELIVERY parameter double; FB1Init70 local boolean =false; FB1ElevDown70 local boolean =false; FB1PistAdv70 local boolean =false; IdenDel local boolean =false; IdenProc local boolean =false; EjectProc local boolean =false; ReturnElev local boolean =false; FB4ElevUp local boolean =false; FB4ElevDown local boolean =false; FB4PistFwd local boolean =false; FB4Air local boolean =false; FB4CartFull local boolean =false; ReqDel local boolean =false; IdenColor local boolean =false; PartOk local boolean =false; EjectOk local boolean =false; PartDiff local boolean =false; EjectBad local boolean =false; FB5ElevUp local boolean =false; FB5ElevDown1 local boolean =false; FB5ElevDown2 local boolean =false; FB5PistFwd1 local boolean =false; FB5PistFwd2 local boolean =false; FB5Air local boolean =false; FB5CartFull local boolean =false; idA70 local boolean =false; idB70 local boolean =false; PartDel70 local boolean =false; RQPartDel70 local boolean =false; RQWrong70 local boolean =false; RQ1_70 local boolean =false; RQ2_70 local boolean =false; RouteOut74 local boolean =false; NoCart74 local boolean =false; CartFull74 local boolean =false; ElevUp70 local boolean =false; ElevDown70 local boolean =false; Eject70 local boolean =false; Air70 local boolean =false; CRouteIn80 local boolean =false; CRouteIn74 local boolean =false; CartStat24 local boolean =false; Optic24 local boolean =false; PistBck24 local boolean =false; ArmMag80 local boolean =false; KeyPos71 local boolean =false; PartToCart local boolean =false; CartHasPart local boolean =false; PartIn70 local boolean =false; ElevLow70 local boolean =false; ElevHigh70 local boolean =false; SInd70 local boolean =false; Height70 local boolean =false; PistBck70 local boolean =false; SStation70 local boolean =false; nTest local double =0; nTestIn local double =0; nReject local double =0; testColor local double =0; tElev local double =0; tPist local double =0; SimActuators_80 output Bus: B_SimActuators_80; SimControl_80 output Bus: B_SimControl_80; SimSensors_80 output Bus: B_SimSensors_80; DIST_MODE parameter double; RQ_PARTS parameter double; MAG_PARTS0 parameter double; MAG_CAP parameter double; T_DIST_T1 parameter double; T_DIST_T2 parameter double; T_DIST_T3 parameter double; T_DIST_T4 parameter double; t_d_a2d_empty parameter double; t_d_a2d_load parameter double; t_d_magoff_empty parameter double; t_d_magoff_load parameter double; t_d_a2m parameter double; t_d_deloff parameter double; t_d_sst_off parameter double; t_d_pist_fwd parameter double; t_d_pist_bckoff parameter double; t_d_pist_back parameter double; t_d_suct parameter double; t_d_release parameter double; DistInit85 local boolean =false; FB1MagEmpty80 local boolean =false; FB1MagFull80 local boolean =false; FB1A2M2_80 local boolean =false; PartinMag80 local boolean =false; PartDel85 local boolean =false; ArmDel80 local boolean =false; PistBck80 local boolean =false; PistFwd80 local boolean =false; PartStuck80 local boolean =false; MagFull80 local boolean =false; MagEmpty80 local boolean =false; KeyPos81 local boolean =false; A2D80 local boolean =false; A2M80 local boolean =false; PistAdv80 local boolean =false; SuctOn80 local boolean =false; SuctOff80 local boolean =false; PartAtPickup local boolean =false; PartInArm local boolean =false; ArmLoaded local boolean =false; prevMagFull80 local boolean =false; prevPistFwd80 local boolean =false; D4On local boolean =false; D4Transport local boolean =false; D4PartStuckM local boolean =false; D4PartDel local boolean =false; D4A2D1 local boolean =false; D4A2D2 local boolean =false; D4A2M1 local boolean =false; D4A2M2 local boolean =false; D4PistFwd local boolean =false; D4SuctOn local boolean =false; D4SuctOff local boolean =false; D5On local boolean =false; D5Transport local boolean =false; D5PartStuckM local boolean =false; D5PartDelEdge local boolean =false; D5A2D1 local boolean =false; D5A2D2 local boolean =false; D5A2M1 local boolean =false; D5A2M2 local boolean =false; D5PistFwd local boolean =false; D5SuctOn local boolean =false; D5SuctOff local boolean =false; D6On local boolean =false; D6Transport local boolean =false; D6PartStuckM local boolean =false; D6PartDel local boolean =false; D6A2D1 local boolean =false; D6A2D2 local boolean =false; D6A2M1 local boolean =false; D6A2M2 local boolean =false; D6PistFwd local boolean =false; D6SuctOn local boolean =false; D6SuctOff local boolean =false; cnt80 local double =0; cnt87 local double =0; magCount local double =0; tArm local double =0; tPistD local double =0; tMagFull local double =0; tMagEmpty local double =0; nDistDel local double =0; SimActuators_100 output Bus: B_SimActuators_100; SimControl_100 output Bus: B_SimControl_100; SimSensors_100 output Bus: B_SimSensors_100; PROC_MODE parameter double; RQ_TURNS parameter double; T_PROC_T4 parameter double; T_PROC_T5 parameter double; T_PROC_T8 parameter double; t_rt_step parameter double; t_rt_hi parameter double; t_ptest_ok parameter double; t_drill_down parameter double; t_drill_up parameter double; PROC_TEST_OK parameter double; ProcInit local boolean =false; P1DrillUp local boolean =false; P1DrillH local boolean =false; P1Empty1 local boolean =false; P1Empty2 local boolean =false; P1RT1 local boolean =false; PartReady100 local boolean =false; PartReadyM local boolean =false; P4Start local boolean =false; P4RT local boolean =false; P4Pin local boolean =false; P4OK local boolean =false; P4Fail local boolean =false; P4Ready local boolean =false; P5Start local boolean =false; P5RT local boolean =false; P5Pin local boolean =false; P5OK local boolean =false; P5Fail local boolean =false; P5DrillPin local boolean =false; P5LDrill local boolean =false; P5TDrill local boolean =false; P5RDrill local boolean =false; P5DrillOk local boolean =false; P5Ready local boolean =false; P6Start local boolean =false; P6RT local boolean =false; P6RotOK local boolean =false; P6Ready local boolean =false; RtOn100 local boolean =false; DrillDown100 local boolean =false; DrillUp100 local boolean =false; DrillPin100 local boolean =false; DrillOn100 local boolean =false; TestPin100 local boolean =false; KeyPos101 local boolean =false; RTSens100 local boolean =false; PInit100 local boolean =false; PTest100 local boolean =false; PDrill100 local boolean =false; SDrillHigh100 local boolean =false; SDrillLow100 local boolean =false; PTestOk100 local boolean =false; PartOnTable local boolean =false; prevRTSens100 local boolean =false; ClawHigh90 local boolean =false; ClawLow90 local boolean =false; ClawDel90 local boolean =false; PartInClaw90 local boolean =false; partOff local double =0; tRt local double =0; cntRT local double =0; cnt106 local double =0; nProcIn local double =0; nProcOut local double =0; procIdx local double =0; SimActuators_90 output Bus: B_SimActuators_90; SimASi_90 output Bus: B_SimASi_90; SimControl_90 output Bus: B_SimControl_90; SimSensors_90 output Bus: B_SimSensors_90; HD2_CART2DEL parameter double; HD2_DEL2CART parameter double; T_HD2_T1 parameter double; T_CONV25_T1 parameter double; t_c2_down parameter double; t_c2_highoff parameter double; t_c2_up parameter double; t_c2_lowoff parameter double; t_c2_2del parameter double; t_c2_2cart parameter double; t_c2_cartoff parameter double; t_c2_deloff parameter double; t_c2_res_del parameter double; t_c2_res_cart parameter double; t_c2_res_dur parameter double; t_c2_grip parameter double; t_c2_open parameter double; t_25_arrive parameter double; t_25_req parameter double; t_25_croute_in0 parameter double; t_25_croute_in parameter double; t_25_pist_bck parameter double; t_25_optic_off parameter double; t_25_leave parameter double; H2Init local boolean =false; H2Arm2Cart local boolean =false; H2ClawHighC local boolean =false; OKMove90 local boolean =false; H4P2D local boolean =false; H4ProcStart local boolean =false; H4Claw2Cart local boolean =false; H4Low1 local boolean =false; H4Close local boolean =false; H4Claw2Del local boolean =false; H4Low2 local boolean =false; H4PartDel local boolean =false; H5P2D local boolean =false; H5ProcStart local boolean =false; H5Claw2Del local boolean =false; H5Low1 local boolean =false; H5Close local boolean =false; H5Claw2Cart local boolean =false; H5Low2 local boolean =false; H5PartDel local boolean =false; ClawDown90 local boolean =false; CloseClaw90 local boolean =false; Claw2Del90 local boolean =false; Claw2Cart90 local boolean =false; ClawCart90 local boolean =false; KeyPos91 local boolean =false; CartStat25 local boolean =false; Optic25 local boolean =false; PistBck25 local boolean =false; CRouteIn94 local boolean =false; RouteOut94 local boolean =false; CartHasPart25 local boolean =false; tC2v local double =0; tC2h local double =0; nCart25 local double =0; nProc25Done local double =0; SimActuators_30 output Bus: B_SimActuators_30; SimASi_30 output Bus: B_SimASi_30; SimControl_30 output Bus: B_SimControl_30; SimSensors_30 output Bus: B_SimSensors_30; SimRFID_RFID output Bus: B_SimRFID_RFID; SimActuators_40 output Bus: B_SimActuators_40; SimASi_40 output Bus: B_SimASi_40; SimControl_40 output Bus: B_SimControl_40; SimSensors_40 output Bus: B_SimSensors_40; ROBOT_MODE parameter double; STOR_MODE parameter double; T_ROB_T7 parameter double; T_ROB_T8 parameter double; T_STOR_T1 parameter double; T_STOR_T2 parameter double; T_STOR_T3 parameter double; T_CONV27_T1 parameter double; T_CONV28_T1 parameter double; t_27_travel parameter double; t_27_optic_stat parameter double; t_27_croute_in0 parameter double; t_27_croute_in parameter double; t_27_pist_bck parameter double; t_27_optic_off parameter double; t_27_leave parameter double; t_28_travel parameter double; t_28_optic_stat parameter double; t_28_croute_in0 parameter double; t_28_croute_in parameter double; t_28_pist_bck parameter double; t_28_optic_off parameter double; t_28_leave parameter double; CartStat27 local boolean =false; Optic27 local boolean =false; CRouteIn34 local boolean =false; RobCartDel local boolean =false; PartDel35 local boolean =false; RouteOut34 local boolean =false; CartStat28 local boolean =false; Optic28 local boolean =false; CRouteIn44 local boolean =false; StorInit local boolean =false; StoreOK local boolean =false; RetrieveOK local boolean =false; ProcessOK44 local boolean =false; RouteOut44 local boolean =false; KeyPos41 local boolean =false; nCart27 local double =0; nCart28 local double =0; nRobDone local double =0; nStorDone local double =0; T_FB11_T parameter double; CART_ID parameter double; t_pin_bck parameter double; t_pin_fwd parameter double; t_cnt_per parameter double; t_cnt_pulse parameter double; t_mes_start parameter double; t_mes_req parameter double; t_opc parameter double; t_mes_reqdur parameter double; t_mes_cri0 parameter double; t_mes_cri parameter double; t_vis parameter double; T_HOP_ARR parameter double; T_HOP_STATOFF parameter double; T_HOP_OPTOFF parameter double; T_HOP_NEXT parameter double; T_HOP_NEXTDUR parameter double; T_OPT_ON parameter double; T_CNT parameter double; CartStat26 local boolean =false; Optic26 local boolean =false; Optic29 local boolean =false; PistBck26 local boolean =false; PistBck27 local boolean =false; PistBck28 local boolean =false; PistBck29 local boolean =false; CartNext24 local boolean =false; CartNext25 local boolean =false; CartNext26 local boolean =false; CartNext27 local boolean =false; CartNext28 local boolean =false; CartNext29 local boolean =false; Count24 local boolean =false; Count25 local boolean =false; Count26 local boolean =false; Count27 local boolean =false; Count28 local boolean =false; Count29 local boolean =false; PinCmd24 local boolean =false; PinCmd25 local boolean =false; PinCmd26 local boolean =false; PinCmd27 local boolean =false; PinCmd28 local boolean =false; PinCmd29 local boolean =false; CRouteIn26 local boolean =false; VisDone26 local boolean =false; RouteOut54 local boolean =false; cartPart local boolean =false; ConvOn22 local boolean =false; ConvErr22 local boolean =false; Selected11 local boolean =false; ControlerOn local boolean =false; MesStart local boolean =false; Req11_Test local boolean =false; Conv11_Test local boolean =false; CartDel11_Test local boolean =false; ReqIn_Test local boolean =false; CTp24 local boolean =false; PBp24 local boolean =false; Path11_Test_Proc local boolean =false; Path11_Test_Visi local boolean =false; Path11_Test_Robo local boolean =false; Path11_Test_Stor local boolean =false; Path11_Test_Sort local boolean =false; Req11_Proc local boolean =false; Conv11_Proc local boolean =false; CartDel11_Proc local boolean =false; ReqIn_Proc local boolean =false; CTp25 local boolean =false; PBp25 local boolean =false; Path11_Proc_Test local boolean =false; Path11_Proc_Visi local boolean =false; Path11_Proc_Robo local boolean =false; Path11_Proc_Stor local boolean =false; Path11_Proc_Sort local boolean =false; Req11_Visi local boolean =false; Conv11_Visi local boolean =false; CartDel11_Visi local boolean =false; ReqIn_Visi local boolean =false; CTp26 local boolean =false; PBp26 local boolean =false; Path11_Visi_Test local boolean =false; Path11_Visi_Proc local boolean =false; Path11_Visi_Robo local boolean =false; Path11_Visi_Stor local boolean =false; Path11_Visi_Sort local boolean =false; Req11_Robo local boolean =false; Conv11_Robo local boolean =false; CartDel11_Robo local boolean =false; ReqIn_Robo local boolean =false; CTp27 local boolean =false; PBp27 local boolean =false; Path11_Robo_Test local boolean =false; Path11_Robo_Proc local boolean =false; Path11_Robo_Visi local boolean =false; Path11_Robo_Stor local boolean =false; Path11_Robo_Sort local boolean =false; Req11_Stor local boolean =false; Conv11_Stor local boolean =false; CartDel11_Stor local boolean =false; ReqIn_Stor local boolean =false; CTp28 local boolean =false; PBp28 local boolean =false; Path11_Stor_Test local boolean =false; Path11_Stor_Proc local boolean =false; Path11_Stor_Visi local boolean =false; Path11_Stor_Robo local boolean =false; Path11_Stor_Sort local boolean =false; Req11_Sort local boolean =false; Conv11_Sort local boolean =false; CartDel11_Sort local boolean =false; ReqIn_Sort local boolean =false; CTp29 local boolean =false; PBp29 local boolean =false; Path11_Sort_Test local boolean =false; Path11_Sort_Proc local boolean =false; Path11_Sort_Visi local boolean =false; Path11_Sort_Robo local boolean =false; Path11_Sort_Stor local boolean =false; cs local double =0; cf local double =0; ct local double =0; tHop local double =0; tcnt local double =0; nLoop local double =0; CID24 local double =0; CID25 local double =0; CID26 local double =0; CID27 local double =0; CID28 local double =0; CID29 local double =0
